simulink model "rfsoc4x2_ospfb_128"  (R2021a)
(part 16 of 339)

      mask prompts: mult_latency "Multiplier Latency"; coeff_width "Coefficient Bit Width In"; coeff_frac_width "Coefficient Fractional Bits"; delay "Data/Sync Delay"; data_width "Data Bit Width In"; bram_latency "BRAM Latency"; use_hdl "Use behavioral HDL for multlipliers"; use_embedded "Use embedded multipliers"
      mask init: same as rfsoc4x2_ospfb_128/pfb_fir_real10/pol1_in1_tap1
  pol1_in1_tap77 : Subsystem  AncestorBlock=casper_library_pfbs/tap_real  mask(pfb_tap_real){mult_latency=2, coeff_width=16, coeff_frac_width=15, delay=16, data_width=16, bram_latency=2, use_hdl=on, use_embedded=off}
      mask prompts: mult_latency "Multiplier Latency"; coeff_width "Coefficient Bit Width In"; coeff_frac_width "Coefficient Fractional Bits"; delay "Data/Sync Delay"; data_width "Data Bit Width In"; bram_latency "BRAM Latency"; use_hdl "Use behavioral HDL for multlipliers"; use_embedded "Use embedded multipliers"
      mask init: same as rfsoc4x2_ospfb_128/pfb_fir_real10/pol1_in1_tap1
  pol1_in1_tap78 : Subsystem  AncestorBlock=casper_library_pfbs/tap_real  mask(pfb_tap_real){mult_latency=2, coeff_width=16, coeff_frac_width=15, delay=16, data_width=16, bram_latency=2, use_hdl=on, use_embedded=off}
      mask prompts: mult_latency "Multiplier Latency"; coeff_width "Coefficient Bit Width In"; coeff_frac_width "Coefficient Fractional Bits"; delay "Data/Sync Delay"; data_width "Data Bit Width In"; bram_latency "BRAM Latency"; use_hdl "Use behavioral HDL for multlipliers"; use_embedded "Use embedded multipliers"
      mask init: same as rfsoc4x2_ospfb_128/pfb_fir_real10/pol1_in1_tap1
  pol1_in1_tap79 : Subsystem  AncestorBlock=casper_library_pfbs/tap_real  mask(pfb_tap_real){mult_latency=2, coeff_width=16, coeff_frac_width=15, delay=16, data_width=16, bram_latency=2, use_hdl=on, use_embedded=off}
      mask prompts: mult_latency "Multiplier Latency"; coeff_width "Coefficient Bit Width In"; coeff_frac_width "Coefficient Fractional Bits"; delay "Data/Sync Delay"; data_width "Data Bit Width In"; bram_latency "BRAM Latency"; use_hdl "Use behavioral HDL for multlipliers"; use_embedded "Use embedded multipliers"
      mask init: same as rfsoc4x2_ospfb_128/pfb_fir_real10/pol1_in1_tap1
  pol1_in1_tap8 : Subsystem  AncestorBlock=casper_library_pfbs/tap_real  mask(pfb_tap_real){mult_latency=2, coeff_width=16, coeff_frac_width=15, delay=16, data_width=16, bram_latency=2, use_hdl=on, use_embedded=off}
      mask prompts: mult_latency "Multiplier Latency"; coeff_width "Coefficient Bit Width In"; coeff_frac_width "Coefficient Fractional Bits"; delay "Data/Sync Delay"; data_width "Data Bit Width In"; bram_latency "BRAM Latency"; use_hdl "Use behavioral HDL for multlipliers"; use_embedded "Use embedded multipliers"
      mask init: same as rfsoc4x2_ospfb_128/pfb_fir_real10/pol1_in1_tap1
  pol1_in1_tap80 : Subsystem  AncestorBlock=casper_library_pfbs/tap_real  mask(pfb_tap_real){mult_latency=2, coeff_width=16, coeff_frac_width=15, delay=16, data_width=16, bram_latency=2, use_hdl=on, use_embedded=off}
      mask prompts: mult_latency "Multiplier Latency"; coeff_width "Coefficient Bit Width In"; coeff_frac_width "Coefficient Fractional Bits"; delay "Data/Sync Delay"; data_width "Data Bit Width In"; bram_latency "BRAM Latency"; use_hdl "Use behavioral HDL for multlipliers"; use_embedded "Use embedded multipliers"
      mask init: same as rfsoc4x2_ospfb_128/pfb_fir_real10/pol1_in1_tap1
  pol1_in1_tap81 : Subsystem  AncestorBlock=casper_library_pfbs/tap_real  mask(pfb_tap_real){mult_latency=2, coeff_width=16, coeff_frac_width=15, delay=16, data_width=16, bram_latency=2, use_hdl=on, use_embedded=off}
      mask prompts: mult_latency "Multiplier Latency"; coeff_width "Coefficient Bit Width In"; coeff_frac_width "Coefficient Fractional Bits"; delay "Data/Sync Delay"; data_width "Data Bit Width In"; bram_latency "BRAM Latency"; use_hdl "Use behavioral HDL for multlipliers"; use_embedded "Use embedded multipliers"
      mask init: same as rfsoc4x2_ospfb_128/pfb_fir_real10/pol1_in1_tap1
  pol1_in1_tap82 : Subsystem  AncestorBlock=casper_library_pfbs/tap_real  mask(pfb_tap_real){mult_latency=2, coeff_width=16, coeff_frac_width=15, delay=16, data_width=16, bram_latency=2, use_hdl=on, use_embedded=off}
      mask prompts: mult_latency "Multiplier Latency"; coeff_width "Coefficient Bit Width In"; coeff_frac_width "Coefficient Fractional Bits"; delay "Data/Sync Delay"; data_width "Data Bit Width In"; bram_latency "BRAM Latency"; use_hdl "Use behavioral HDL for multlipliers"; use_embedded "Use embedded multipliers"
      mask init: same as rfsoc4x2_ospfb_128/pfb_fir_real10/pol1_in1_tap1
  pol1_in1_tap83 : Subsystem  AncestorBlock=casper_library_pfbs/tap_real  mask(pfb_tap_real){mult_latency=2, coeff_width=16, coeff_frac_width=15, delay=16, data_width=16, bram_latency=2, use_hdl=on, use_embedded=off}
      mask prompts: mult_latency "Multiplier Latency"; coeff_width "Coefficient Bit Width In"; coeff_frac_width "Coefficient Fractional Bits"; delay "Data/Sync Delay"; data_width "Data Bit Width In"; bram_latency "BRAM Latency"; use_hdl "Use behavioral HDL for multlipliers"; use_embedded "Use embedded multipliers"
      mask init: same as rfsoc4x2_ospfb_128/pfb_fir_real10/pol1_in1_tap1
  pol1_in1_tap84 : Subsystem  AncestorBlock=casper_library_pfbs/tap_real  mask(pfb_tap_real){mult_latency=2, coeff_width=16, coeff_frac_width=15, delay=16, data_width=16, bram_latency=2, use_hdl=on, use_embedded=off}
      mask prompts: mult_latency "Multiplier Latency"; coeff_width "Coefficient Bit Width In"; coeff_frac_width "Coefficient Fractional Bits"; delay "Data/Sync Delay"; data_width "Data Bit Width In"; bram_latency "BRAM Latency"; use_hdl "Use behavioral HDL for multlipliers"; use_embedded "Use embedded multipliers"
      mask init: same as rfsoc4x2_ospfb_128/pfb_fir_real10/pol1_in1_tap1
  pol1_in1_tap85 : Subsystem  AncestorBlock=casper_library_pfbs/tap_real  mask(pfb_tap_real){mult_latency=2, coeff_width=16, coeff_frac_width=15, delay=16, data_width=16, bram_latency=2, use_hdl=on, use_embedded=off}
      mask prompts: mult_latency "Multiplier Latency"; coeff_width "Coefficient Bit Width In"; coeff_frac_width "Coefficient Fractional Bits"; delay "Data/Sync Delay"; data_width "Data Bit Width In"; bram_latency "BRAM Latency"; use_hdl "Use behavioral HDL for multlipliers"; use_embedded "Use embedded multipliers"
      mask init: same as rfsoc4x2_ospfb_128/pfb_fir_real10/pol1_in1_tap1
  pol1_in1_tap86 : Subsystem  AncestorBlock=casper_library_pfbs/tap_real  mask(pfb_tap_real){mult_latency=2, coeff_width=16, coeff_frac_width=15, delay=16, data_width=16, bram_latency=2, use_hdl=on, use_embedded=off}
      mask prompts: mult_latency "Multiplier Latency"; coeff_width "Coefficient Bit Width In"; coeff_frac_width "Coefficient Fractional Bits"; delay "Data/Sync Delay"; data_width "Data Bit Width In"; bram_latency "BRAM Latency"; use_hdl "Use behavioral HDL for multlipliers"; use_embedded "Use embedded multipliers"
      mask init: same as rfsoc4x2_ospfb_128/pfb_fir_real10/pol1_in1_tap1
  pol1_in1_tap87 : Subsystem  AncestorBlock=casper_library_pfbs/tap_real  mask(pfb_tap_real){mult_latency=2, coeff_width=16, coeff_frac_width=15, delay=16, data_width=16, bram_latency=2, use_hdl=on, use_embedded=off}
      mask prompts: mult_latency "Multiplier Latency"; coeff_width "Coefficient Bit Width In"; coeff_frac_width "Coefficient Fractional Bits"; delay "Data/Sync Delay"; data_width "Data Bit Width In"; bram_latency "BRAM Latency"; use_hdl "Use behavioral HDL for multlipliers"; use_embedded "Use embedded multipliers"
      mask init: same as rfsoc4x2_ospfb_128/pfb_fir_real10/pol1_in1_tap1
  pol1_in1_tap88 : Subsystem  AncestorBlock=casper_library_pfbs/tap_real  mask(pfb_tap_real){mult_latency=2, coeff_width=16, coeff_frac_width=15, delay=16, data_width=16, bram_latency=2, use_hdl=on, use_embedded=off}
      mask prompts: mult_latency "Multiplier Latency"; coeff_width "Coefficient Bit Width In"; coeff_frac_width "Coefficient Fractional Bits"; delay "Data/Sync Delay"; data_width "Data Bit Width In"; bram_latency "BRAM Latency"; use_hdl "Use behavioral HDL for multlipliers"; use_embedded "Use embedded multipliers"
      mask init: same as rfsoc4x2_ospfb_128/pfb_fir_real10/pol1_in1_tap1
  pol1_in1_tap89 : Subsystem  AncestorBlock=casper_library_pfbs/tap_real  mask(pfb_tap_real){mult_latency=2, coeff_width=16, coeff_frac_width=15, delay=16, data_width=16, bram_latency=2, use_hdl=on, use_embedded=off}
      mask prompts: mult_latency "Multiplier Latency"; coeff_width "Coefficient Bit Width In"; coeff_frac_width "Coefficient Fractional Bits"; delay "Data/Sync Delay"; data_width "Data Bit Width In"; bram_latency "BRAM Latency"; use_hdl "Use behavioral HDL for multlipliers"; use_embedded "Use embedded multipliers"
      mask init: same as rfsoc4x2_ospfb_128/pfb_fir_real10/pol1_in1_tap1
  pol1_in1_tap9 : Subsystem  AncestorBlock=casper_library_pfbs/tap_real  mask(pfb_tap_real){mult_latency=2, coeff_width=16, coeff_frac_width=15, delay=16, data_width=16, bram_latency=2, use_hdl=on, use_embedded=off}
      mask prompts: mult_latency "Multiplier Latency"; coeff_width "Coefficient Bit Width In"; coeff_frac_width "Coefficient Fractional Bits"; delay "Data/Sync Delay"; data_width "Data Bit Width In"; bram_latency "BRAM Latency"; use_hdl "Use behavioral HDL for multlipliers"; use_embedded "Use embedded multipliers"
      mask init: same as rfsoc4x2_ospfb_128/pfb_fir_real10/pol1_in1_tap1
  pol1_in1_tap90 : Subsystem  AncestorBlock=casper_library_pfbs/tap_real  mask(pfb_tap_real){mult_latency=2, coeff_width=16, coeff_frac_width=15, delay=16, data_width=16, bram_latency=2, use_hdl=on, use_embedded=off}
      mask prompts: mult_latency "Multiplier Latency"; coeff_width "Coefficient Bit Width In"; coeff_frac_width "Coefficient Fractional Bits"; delay "Data/Sync Delay"; data_width "Data Bit Width In"; bram_latency "BRAM Latency"; use_hdl "Use behavioral HDL for multlipliers"; use_embedded "Use embedded multipliers"
      mask init: same as rfsoc4x2_ospfb_128/pfb_fir_real10/pol1_in1_tap1
  pol1_in1_tap91 : Subsystem  AncestorBlock=casper_library_pfbs/tap_real  mask(pfb_tap_real){mult_latency=2, coeff_width=16, coeff_frac_width=15, delay=16, data_width=16, bram_latency=2, use_hdl=on, use_embedded=off}
      mask prompts: mult_latency "Multiplier Latency"; coeff_width "Coefficient Bit Width In"; coeff_frac_width "Coefficient Fractional Bits"; delay "Data/Sync Delay"; data_width "Data Bit Width In"; bram_latency "BRAM Latency"; use_hdl "Use behavioral HDL for multlipliers"; use_embedded "Use embedded multipliers"
      mask init: same as rfsoc4x2_ospfb_128/pfb_fir_real10/pol1_in1_tap1
  pol1_in1_tap92 : Subsystem  AncestorBlock=casper_library_pfbs/tap_real  mask(pfb_tap_real){mult_latency=2, coeff_width=16, coeff_frac_width=15, delay=16, data_width=16, bram_latency=2, use_hdl=on, use_embedded=off}
      mask prompts: mult_latency "Multiplier Latency"; coeff_width "Coefficient Bit Width In"; coeff_frac_width "Coefficient Fractional Bits"; delay "Data/Sync Delay"; data_width "Data Bit Width In"; bram_latency "BRAM Latency"; use_hdl "Use behavioral HDL for multlipliers"; use_embedded "Use embedded multipliers"
      mask init: same as rfsoc4x2_ospfb_128/pfb_fir_real10/pol1_in1_tap1
  pol1_in1_tap93 : Subsystem  AncestorBlock=casper_library_pfbs/tap_real  mask(pfb_tap_real){mult_latency=2, coeff_width=16, coeff_frac_width=15, delay=16, data_width=16, bram_latency=2, use_hdl=on, use_embedded=off}
      mask prompts: mult_latency "Multiplier Latency"; coeff_width "Coefficient Bit Width In"; coeff_frac_width "Coefficient Fractional Bits"; delay "Data/Sync Delay"; data_width "Data Bit Width In"; bram_latency "BRAM Latency"; use_hdl "Use behavioral HDL for multlipliers"; use_embedded "Use embedded multipliers"
      mask init: same as rfsoc4x2_ospfb_128/pfb_fir_real10/pol1_in1_tap1
  pol1_in1_tap94 : Subsystem  AncestorBlock=casper_library_pfbs/tap_real  mask(pfb_tap_real){mult_latency=2, coeff_width=16, coeff_frac_width=15, delay=16, data_width=16, bram_latency=2, use_hdl=on, use_embedded=off}
      mask prompts: mult_latency "Multiplier Latency"; coeff_width "Coefficient Bit Width In"; coeff_frac_width "Coefficient Fractional Bits"; delay "Data/Sync Delay"; data_width "Data Bit Width In"; bram_latency "BRAM Latency"; use_hdl "Use behavioral HDL for multlipliers"; use_embedded "Use embedded multipliers"
      mask init: same as rfsoc4x2_ospfb_128/pfb_fir_real10/pol1_in1_tap1
  pol1_in1_tap95 : Subsystem  AncestorBlock=casper_library_pfbs/tap_real  mask(pfb_tap_real){mult_latency=2, coeff_width=16, coeff_frac_width=15, delay=16, data_width=16, bram_latency=2, use_hdl=on, use_embedded=off}
      mask prompts: mult_latency "Multiplier Latency"; coeff_width "Coefficient Bit Width In"; coeff_frac_width "Coefficient Fractional Bits"; delay "Data/Sync Delay"; data_width "Data Bit Width In"; bram_latency "BRAM Latency"; use_hdl "Use behavioral HDL for multlipliers"; use_embedded "Use embedded multipliers"
      mask init: same as rfsoc4x2_ospfb_128/pfb_fir_real10/pol1_in1_tap1
  pol1_in1_tap96 : Subsystem  AncestorBlock=casper_library_pfbs/tap_real  mask(pfb_tap_real){mult_latency=2, coeff_width=16, coeff_frac_width=15, delay=16, data_width=16, bram_latency=2, use_hdl=on, use_embedded=off}
      mask prompts: mult_latency "Multiplier Latency"; coeff_width "Coefficient Bit Width In"; coeff_frac_width "Coefficient Fractional Bits"; delay "Data/Sync Delay"; data_width "Data Bit Width In"; bram_latency "BRAM Latency"; use_hdl "Use behavioral HDL for multlipliers"; use_embedded "Use embedded multipliers"
      mask init: same as rfsoc4x2_ospfb_128/pfb_fir_real10/pol1_in1_tap1
  pol1_in2_coeffs : Subsystem  AncestorBlock=casper_library_pfbs/pfb_coeff_gen  mask(pfb_coeff_gen){PFBSize=8, CoeffBitWidth=16, TotalTaps=8, CoeffDistMem=off, WindowType=hamming, bram_latency=2, n_inputs=4, nput=1, fwidth=1.245000000000000106581410364015, debug_mode=off, fan_latency=1}
      mask prompts: PFBSize "Size of PFB: (2^? pnts)"; CoeffBitWidth "Bitwidth of Coefficients:"; TotalTaps "Total Number of Taps:"; CoeffDistMem "Implement Coeff Gen in Distributed Memory"; WindowType "Windowing Function:"; bram_latency "BRAM Latency"; n_inputs "Number of Simultaneous Inputs: (2^?)"; nput "This is input number:"; fwidth "Bin Width (normal=1)"; debug_mode "Debug mode - coeffs are a [1:pfb_size*taps] ramp."; fan_latency "Fanout latency"
      mask init: same as rfsoc4x2_ospfb_128/pfb_fir_real10/pol1_in10_coeffs
      settings: AttributesFormatString=|
      | PFBSize=8, n_inputs=4,
      | taps=8, input=1
  pol1_in3_coeffs : Subsystem  AncestorBlock=casper_library_pfbs/pfb_coeff_gen  mask(pfb_coeff_gen){PFBSize=8, CoeffBitWidth=16, TotalTaps=8, CoeffDistMem=off, WindowType=hamming, bram_latency=2, n_inputs=4, nput=2, fwidth=1.245000000000000106581410364015, debug_mode=off, fan_latency=1}
      mask prompts: PFBSize "Size of PFB: (2^? pnts)"; CoeffBitWidth "Bitwidth of Coefficients:"; TotalTaps "Total Number of Taps:"; CoeffDistMem "Implement Coeff Gen in Distributed Memory"; WindowType "Windowing Function:"; bram_latency "BRAM Latency"; n_inputs "Number of Simultaneous Inputs: (2^?)"; nput "This is input number:"; fwidth "Bin Width (normal=1)"; debug_mode "Debug mode - coeffs are a [1:pfb_size*taps] ramp."; fan_latency "Fanout latency"
      mask init: same as rfsoc4x2_ospfb_128/pfb_fir_real10/pol1_in10_coeffs
      settings: AttributesFormatString=|
      | PFBSize=8, n_inputs=4,
      | taps=8, input=2
  pol1_in4_coeffs : Subsystem  AncestorBlock=casper_library_pfbs/pfb_coeff_gen  mask(pfb_coeff_gen){PFBSize=8, CoeffBitWidth=16, TotalTaps=8, CoeffDistMem=off, WindowType=hamming, bram_latency=2, n_inputs=4, nput=3, fwidth=1.245000000000000106581410364015, debug_mode=off, fan_latency=1}
      mask prompts: PFBSize "Size of PFB: (2^? pnts)"; CoeffBitWidth "Bitwidth of Coefficients:"; TotalTaps "Total Number of Taps:"; CoeffDistMem "Implement Coeff Gen in Distributed Memory"; WindowType "Windowing Function:"; bram_latency "BRAM Latency"; n_inputs "Number of Simultaneous Inputs: (2^?)"; nput "This is input number:"; fwidth "Bin Width (normal=1)"; debug_mode "Debug mode - coeffs are a [1:pfb_size*taps] ramp."; fan_latency "Fanout latency"
      mask init: same as rfsoc4x2_ospfb_128/pfb_fir_real10/pol1_in10_coeffs
      settings: AttributesFormatString=|
      | PFBSize=8, n_inputs=4,
      | taps=8, input=3
  pol1_in5_coeffs : Subsystem  AncestorBlock=casper_library_pfbs/pfb_coeff_gen  mask(pfb_coeff_gen){PFBSize=8, CoeffBitWidth=16, TotalTaps=8, CoeffDistMem=off, WindowType=hamming, bram_latency=2, n_inputs=4, nput=4, fwidth=1.245000000000000106581410364015, debug_mode=off, fan_latency=1}
      mask prompts: PFBSize "Size of PFB: (2^? pnts)"; CoeffBitWidth "Bitwidth of Coefficients:"; TotalTaps "Total Number of Taps:"; CoeffDistMem "Implement Coeff Gen in Distributed Memory"; WindowType "Windowing Function:"; bram_latency "BRAM Latency"; n_inputs "Number of Simultaneous Inputs: (2^?)"; nput "This is input number:"; fwidth "Bin Width (normal=1)"; debug_mode "Debug mode - coeffs are a [1:pfb_size*taps] ramp."; fan_latency "Fanout latency"
      mask init: same as rfsoc4x2_ospfb_128/pfb_fir_real10/pol1_in10_coeffs
      settings: AttributesFormatString=|
      | PFBSize=8, n_inputs=4,
      | taps=8, input=4
  pol1_in6_coeffs : Subsystem  AncestorBlock=casper_library_pfbs/pfb_coeff_gen  mask(pfb_coeff_gen){PFBSize=8, CoeffBitWidth=16, TotalTaps=8, CoeffDistMem=off, WindowType=hamming, bram_latency=2, n_inputs=4, nput=5, fwidth=1.245000000000000106581410364015, debug_mode=off, fan_latency=1}
      mask prompts: PFBSize "Size of PFB: (2^? pnts)"; CoeffBitWidth "Bitwidth of Coefficients:"; TotalTaps "Total Number of Taps:"; CoeffDistMem "Implement Coeff Gen in Distributed Memory"; WindowType "Windowing Function:"; bram_latency "BRAM Latency"; n_inputs "Number of Simultaneous Inputs: (2^?)"; nput "This is input number:"; fwidth "Bin Width (normal=1)"; debug_mode "Debug mode - coeffs are a [1:pfb_size*taps] ramp."; fan_latency "Fanout latency"
      mask init: same as rfsoc4x2_ospfb_128/pfb_fir_real10/pol1_in10_coeffs
      settings: AttributesFormatString=|
      | PFBSize=8, n_inputs=4,
      | taps=8, input=5
  pol1_in7_coeffs : Subsystem  AncestorBlock=casper_library_pfbs/pfb_coeff_gen  mask(pfb_coeff_gen){PFBSize=8, CoeffBitWidth=16, TotalTaps=8, CoeffDistMem=off, WindowType=hamming, bram_latency=2, n_inputs=4, nput=6, fwidth=1.245000000000000106581410364015, debug_mode=off, fan_latency=1}
      mask prompts: PFBSize "Size of PFB: (2^? pnts)"; CoeffBitWidth "Bitwidth of Coefficients:"; TotalTaps "Total Number of Taps:"; CoeffDistMem "Implement Coeff Gen in Distributed Memory"; WindowType "Windowing Function:"; bram_latency "BRAM Latency"; n_inputs "Number of Simultaneous Inputs: (2^?)"; nput "This is input number:"; fwidth "Bin Width (normal=1)"; debug_mode "Debug mode - coeffs are a [1:pfb_size*taps] ramp."; fan_latency "Fanout latency"
      mask init: same as rfsoc4x2_ospfb_128/pfb_fir_real10/pol1_in10_coeffs
      settings: AttributesFormatString=|
      | PFBSize=8, n_inputs=4,
      | taps=8, input=6
  pol1_in8_coeffs : Subsystem  AncestorBlock=casper_library_pfbs/pfb_coeff_gen  mask(pfb_coeff_gen){PFBSize=8, CoeffBitWidth=16, TotalTaps=8, CoeffDistMem=off, WindowType=hamming, bram_latency=2, n_inputs=4, nput=7, fwidth=1.245000000000000106581410364015, debug_mode=off, fan_latency=1}
      mask prompts: PFBSize "Size of PFB: (2^? pnts)"; CoeffBitWidth "Bitwidth of Coefficients:"; TotalTaps "Total Number of Taps:"; CoeffDistMem "Implement Coeff Gen in Distributed Memory"; WindowType "Windowing Function:"; bram_latency "BRAM Latency"; n_inputs "Number of Simultaneous Inputs: (2^?)"; nput "This is input number:"; fwidth "Bin Width (normal=1)"; debug_mode "Debug mode - coeffs are a [1:pfb_size*taps] ramp."; fan_latency "Fanout latency"
      mask init: same as rfsoc4x2_ospfb_128/pfb_fir_real10/pol1_in10_coeffs
      settings: AttributesFormatString=|
      | PFBSize=8, n_inputs=4,
      | taps=8, input=7
  pol1_in9_coeffs : Subsystem  AncestorBlock=casper_library_pfbs/pfb_coeff_gen  mask(pfb_coeff_gen){PFBSize=8, CoeffBitWidth=16, TotalTaps=8, CoeffDistMem=off, WindowType=hamming, bram_latency=2, n_inputs=4, nput=8, fwidth=1.245000000000000106581410364015, debug_mode=off, fan_latency=1}
      mask prompts: PFBSize "Size of PFB: (2^? pnts)"; CoeffBitWidth "Bitwidth of Coefficients:"; TotalTaps "Total Number of Taps:"; CoeffDistMem "Implement Coeff Gen in Distributed Memory"; WindowType "Windowing Function:"; bram_latency "BRAM Latency"; n_inputs "Number of Simultaneous Inputs: (2^?)"; nput "This is input number:"; fwidth "Bin Width (normal=1)"; debug_mode "Debug mode - coeffs are a [1:pfb_size*taps] ramp."; fan_latency "Fanout latency"
      mask init: same as rfsoc4x2_ospfb_128/pfb_fir_real10/pol1_in10_coeffs
      settings: AttributesFormatString=|
      | PFBSize=8, n_inputs=4,
      | taps=8, input=8
  scale_1_{1..16} (16 alike) : xbsIndex_r4/Scale  scale_factor=-1  dbl_ovrd=off  block_type=scale
  scope{85..86,88..90} (5 alike) : Scope
  sync_out : Outport  VectorParamsAs1DForOutWhenUnconnected=off
  pol1_out1 : Outport  Port=2  VectorParamsAs1DForOutWhenUnconnected=off
  pol1_out2 : Outport  Port=3  VectorParamsAs1DForOutWhenUnconnected=off
  pol1_out3 : Outport  Port=4
  pol1_out4 : Outport  Port=5
  pol1_out5 : Outport  Port=6
  pol1_out6 : Outport  Port=7
  pol1_out7 : Outport  Port=8
  pol1_out8 : Outport  Port=9
  pol1_out9 : Outport  Port=10
  pol1_out10 : Outport  Port=11
  pol1_out11 : Outport  Port=12
  pol1_out12 : Outport  Port=13
  pol1_out13 : Outport  Port=14
  pol1_out14 : Outport  Port=15
  pol1_out15 : Outport  Port=16
  pol1_out16 : Outport  Port=17
  wires:
  pol1_in1_last_tap/1(tap_out) -> adder_1_1/9(din8)
  delay25/1 -> adder_1_1/1(sync)
  pol1_in1_last_tap/2(sync_out) -> delay25/1
  delay24/1 -> adder_1_1/2(din1)
  delay23/1 -> adder_1_1/3(din2)
  delay22/1 -> adder_1_1/4(din3)
  delay21/1 -> adder_1_1/5(din4)
  delay20/1 -> adder_1_1/6(din5)
  delay19/1 -> adder_1_1/7(din6)
  delay18/1 -> adder_1_1/8(din7)
  pol1_in1_tap3/1(dout) -> pol1_in1_tap4/1(din)
  pol1_in1_tap6/6(pot_en_out) -> pol1_in1_tap7/5(pot_en_in)
  pol1_in1_tap6/5(add_out) -> pol1_in1_tap7/4(addr_in)
  pol1_in1_tap5/6(pot_en_out) -> pol1_in1_tap6/5(pot_en_in)
  pol1_in1_tap5/5(add_out) -> pol1_in1_tap6/4(addr_in)
  pol1_in1_tap4/6(pot_en_out) -> pol1_in1_tap5/5(pot_en_in)
  pol1_in1_tap4/5(add_out) -> pol1_in1_tap5/4(addr_in)
  pol1_in1_tap3/6(pot_en_out) -> pol1_in1_tap4/5(pot_en_in)
  pol1_in1_tap3/5(add_out) -> pol1_in1_tap4/4(addr_in)
  pol1_in1_tap2/6(pot_en_out) -> pol1_in1_tap3/5(pot_en_in)
  pol1_in1_tap2/5(add_out) -> pol1_in1_tap3/4(addr_in)
  pol1_in1_first_tap/6(pot_en_out) -> pol1_in1_tap2/5(pot_en_in)
  pol1_in1_first_tap/5(add_out) -> pol1_in1_tap2/4(addr_in)
  [tap_write_en] -> pol1_in1_first_tap/5(pot_en_in)
  [addr] -> pol1_in1_first_tap/4(addr_in)
  Inverter/1 -> [tap_write_en], Gateway Out255/1
  sync/1 -> pol1_in16_coeffs/2(sync), pol1_in15_coeffs/2(sync), pol1_in14_coeffs/2(sync), pol1_in13_coeffs/2(sync), pol1_in12_coeffs/2(sync), pol1_in11_coeffs/2(sync), pol1_in10_coeffs/2(sync), pol1_in9_coeffs/2(sync), pol1_in8_coeffs/2(sync), pol1_in7_coeffs/2(sync), pol1_in6_coeffs/2(sync), pol1_in5_coeffs/2(sync), pol1_in4_coeffs/2(sync), pol1_in3_coeffs/2(sync), pol1_in2_coeffs/2(sync), pol1_in1_coeffs/2(sync), delay2/1
  AddSub12/1 -> Mux3/3
  Mux3/1 -> [addr], Gateway Out251/1
  edge_detect8/1(out) -> Logical11/2
  Delay27/1 -> Logical11/1
  Counter36/1 -> AddSub11/2, Gateway Out253/1
  Constant61/1 -> Relational11/2
  Constant63/1 -> Relational12/2
  Slice20/1 -> edge_detect8/1(in)
  AddSub11/1 -> AddSub12/1, Mux3/2, Relational11/1, Gateway Out250/1
  Constant62/1 -> AddSub12/2
  Counter38/1 -> Slice20/1, Delay26/1
  Relational11/1 -> Mux3/1
  delay2/1 -> Counter36/1, Counter38/1
  Relational12/1 -> Inverter/1
  Delay26/1 -> Relational12/1, AddSub11/1, Gateway Out252/1
  Logical11/1 -> Counter36/2
  Gateway Out251/1 -> scope86/1
  Gateway Out255/1 -> scope90/1
  Gateway Out250/1 -> scope89/1
  en_ctrl/1 -> Delay27/1
  Gateway Out253/1 -> scope85/1
  Gateway Out252/1 -> scope88/1
  pol1_in1_tap7/4(taps_out) -> delay18/1
  pol1_in1_tap7/3(coeff_out) -> pol1_in1_last_tap/3(coeff)
  pol1_in1_tap7/2(sync_out) -> pol1_in1_last_tap/2(sync)
  pol1_in1_tap7/1(dout) -> pol1_in1_last_tap/1(din)
  pol1_in1_tap6/4(taps_out) -> delay19/1
  pol1_in1_tap6/3(coeff_out) -> pol1_in1_tap7/3(coeff)
  pol1_in1_tap6/2(sync_out) -> pol1_in1_tap7/2(sync)
  pol1_in1_tap6/1(dout) -> pol1_in1_tap7/1(din)
  pol1_in1_tap5/4(taps_out) -> delay20/1
  pol1_in1_tap5/3(coeff_out) -> pol1_in1_tap6/3(coeff)
  pol1_in1_tap5/2(sync_out) -> pol1_in1_tap6/2(sync)
  pol1_in1_tap5/1(dout) -> pol1_in1_tap6/1(din)
  pol1_in1_tap4/4(taps_out) -> delay21/1
  pol1_in1_tap4/3(coeff_out) -> pol1_in1_tap5/3(coeff)
  pol1_in1_tap4/2(sync_out) -> pol1_in1_tap5/2(sync)
  pol1_in1_tap4/1(dout) -> pol1_in1_tap5/1(din)
  pol1_in1_tap3/4(taps_out) -> delay22/1
  pol1_in1_tap3/3(coeff_out) -> pol1_in1_tap4/3(coeff)
  pol1_in1_tap3/2(sync_out) -> pol1_in1_tap4/2(sync)
  pol1_in1_tap2/4(taps_out) -> delay23/1
  pol1_in1_tap2/3(coeff_out) -> pol1_in1_tap3/3(coeff)
  pol1_in1_tap2/2(sync_out) -> pol1_in1_tap3/2(sync)
  pol1_in1_tap2/1(dout) -> pol1_in1_tap3/1(din)
  pol1_in1_first_tap/4(taps_out) -> delay24/1
  pol1_in1_first_tap/3(coeff_out) -> pol1_in1_tap2/3(coeff)
  pol1_in1_first_tap/2(sync_out) -> pol1_in1_tap2/2(sync)
  pol1_in1_first_tap/1(dout) -> pol1_in1_tap2/1(din)
  convert_1_16/1 -> pol1_out16/1
  scale_1_16/1 -> convert_1_16/1
  adder_1_16/2(dout) -> scale_1_16/1
  convert_1_15/1 -> pol1_out15/1
  scale_1_15/1 -> convert_1_15/1
  adder_1_15/2(dout) -> scale_1_15/1
  convert_1_14/1 -> pol1_out14/1
  scale_1_14/1 -> convert_1_14/1
  adder_1_14/2(dout) -> scale_1_14/1
  convert_1_13/1 -> pol1_out13/1
  scale_1_13/1 -> convert_1_13/1
  adder_1_13/2(dout) -> scale_1_13/1
  convert_1_12/1 -> pol1_out12/1
  scale_1_12/1 -> convert_1_12/1
  adder_1_12/2(dout) -> scale_1_12/1
  convert_1_11/1 -> pol1_out11/1
  scale_1_11/1 -> convert_1_11/1
  adder_1_11/2(dout) -> scale_1_11/1
  convert_1_10/1 -> pol1_out10/1
  scale_1_10/1 -> convert_1_10/1
  adder_1_10/2(dout) -> scale_1_10/1
  convert_1_9/1 -> pol1_out9/1
  scale_1_9/1 -> convert_1_9/1
  adder_1_9/2(dout) -> scale_1_9/1
  convert_1_8/1 -> pol1_out8/1
  scale_1_8/1 -> convert_1_8/1
  adder_1_8/2(dout) -> scale_1_8/1
  convert_1_7/1 -> pol1_out7/1
  scale_1_7/1 -> convert_1_7/1
  adder_1_7/2(dout) -> scale_1_7/1
  convert_1_6/1 -> pol1_out6/1
  scale_1_6/1 -> convert_1_6/1
  adder_1_6/2(dout) -> scale_1_6/1
  convert_1_5/1 -> pol1_out5/1
  scale_1_5/1 -> convert_1_5/1
  adder_1_5/2(dout) -> scale_1_5/1
  convert_1_4/1 -> pol1_out4/1
  scale_1_4/1 -> convert_1_4/1
  adder_1_4/2(dout) -> scale_1_4/1
  convert_1_3/1 -> pol1_out3/1
  scale_1_3/1 -> convert_1_3/1
  adder_1_3/2(dout) -> scale_1_3/1
  convert_1_2/1 -> pol1_out2/1
  scale_1_2/1 -> convert_1_2/1
  adder_1_2/2(dout) -> scale_1_2/1
  convert_1_1/1 -> pol1_out1/1
  scale_1_1/1 -> convert_1_1/1
  adder_1_1/2(dout) -> scale_1_1/1
  delay1/1 -> sync_out/1
  adder_1_1/1(sync_out) -> delay1/1
  pol1_in16/1 -> pol1_in16_coeffs/1(din)
  pol1_in15/1 -> pol1_in15_coeffs/1(din)
  pol1_in14/1 -> pol1_in14_coeffs/1(din)
  pol1_in13/1 -> pol1_in13_coeffs/1(din)
  pol1_in12/1 -> pol1_in12_coeffs/1(din)
  pol1_in11/1 -> pol1_in11_coeffs/1(din)
  pol1_in10/1 -> pol1_in10_coeffs/1(din)
  pol1_in9/1 -> pol1_in9_coeffs/1(din)
  pol1_in8/1 -> pol1_in8_coeffs/1(din)
  pol1_in7/1 -> pol1_in7_coeffs/1(din)
  pol1_in6/1 -> pol1_in6_coeffs/1(din)
  pol1_in5/1 -> pol1_in5_coeffs/1(din)
  pol1_in4/1 -> pol1_in4_coeffs/1(din)
  pol1_in3/1 -> pol1_in3_coeffs/1(din)
  pol1_in2/1 -> pol1_in2_coeffs/1(din)
  pol1_in1_coeffs/3(coeff) -> pol1_in1_first_tap/3(coeffs)
  pol1_in1_coeffs/1(dout) -> pol1_in1_first_tap/1(din)
  pol1_in1/1 -> pol1_in1_coeffs/1(din)
  pol1_in1_coeffs/2(sync_out) -> pol1_in1_first_tap/2(sync)
  pol1_in1_first_tap1/1(dout) -> pol1_in1_tap1/1(din)
  pol1_in1_first_tap1/2(sync_out) -> pol1_in1_tap1/2(sync)
  pol1_in1_first_tap1/3(coeff_out) -> pol1_in1_tap1/3(coeff)
  pol1_in1_first_tap1/4(taps_out) -> delay9/1
  pol1_in1_tap1/1(dout) -> pol1_in1_tap8/1(din)
  pol1_in1_tap1/2(sync_out) -> pol1_in1_tap8/2(sync)
  pol1_in1_tap1/3(coeff_out) -> pol1_in1_tap8/3(coeff)
  pol1_in1_tap1/4(taps_out) -> delay8/1
  pol1_in1_tap8/2(sync_out) -> pol1_in1_tap9/2(sync)
  pol1_in1_tap8/3(coeff_out) -> pol1_in1_tap9/3(coeff)
  pol1_in1_tap8/4(taps_out) -> delay7/1
  pol1_in1_tap9/1(dout) -> pol1_in1_tap10/1(din)
  pol1_in1_tap9/2(sync_out) -> pol1_in1_tap10/2(sync)
  pol1_in1_tap9/3(coeff_out) -> pol1_in1_tap10/3(coeff)
  pol1_in1_tap9/4(taps_out) -> delay6/1
  pol1_in1_tap10/1(dout) -> pol1_in1_tap11/1(din)
  pol1_in1_tap10/2(sync_out) -> pol1_in1_tap11/2(sync)
  pol1_in1_tap10/3(coeff_out) -> pol1_in1_tap11/3(coeff)
  pol1_in1_tap10/4(taps_out) -> delay5/1
  pol1_in1_tap11/1(dout) -> pol1_in1_tap12/1(din)
  pol1_in1_tap11/2(sync_out) -> pol1_in1_tap12/2(sync)
  pol1_in1_tap11/3(coeff_out) -> pol1_in1_tap12/3(coeff)
  pol1_in1_tap11/4(taps_out) -> delay4/1
  pol1_in1_tap12/1(dout) -> pol1_in1_last_tap1/1(din)
  pol1_in1_tap12/2(sync_out) -> pol1_in1_last_tap1/2(sync)
  pol1_in1_tap12/3(coeff_out) -> pol1_in1_last_tap1/3(coeff)
  pol1_in1_tap12/4(taps_out) -> delay3/1
  pol1_in1_first_tap1/5(add_out) -> pol1_in1_tap1/4(addr_in)
  pol1_in1_first_tap1/6(pot_en_out) -> pol1_in1_tap1/5(pot_en_in)
  pol1_in1_tap1/5(add_out) -> pol1_in1_tap8/4(addr_in)
  pol1_in1_tap1/6(pot_en_out) -> pol1_in1_tap8/5(pot_en_in)
  pol1_in1_tap8/5(add_out) -> pol1_in1_tap9/4(addr_in)
  pol1_in1_tap8/6(pot_en_out) -> pol1_in1_tap9/5(pot_en_in)
  pol1_in1_tap9/5(add_out) -> pol1_in1_tap10/4(addr_in)
  pol1_in1_tap9/6(pot_en_out) -> pol1_in1_tap10/5(pot_en_in)
  pol1_in1_tap10/5(add_out) -> pol1_in1_tap11/4(addr_in)
  pol1_in1_tap10/6(pot_en_out) -> pol1_in1_tap11/5(pot_en_in)
  pol1_in1_tap11/5(add_out) -> pol1_in1_tap12/4(addr_in)
  pol1_in1_tap11/6(pot_en_out) -> pol1_in1_tap12/5(pot_en_in)
  pol1_in1_tap8/1(dout) -> pol1_in1_tap9/1(din)
  delay3/1 -> adder_1_2/8(din7)
  delay4/1 -> adder_1_2/7(din6)
  delay5/1 -> adder_1_2/6(din5)
  delay6/1 -> adder_1_2/5(din4)
  delay7/1 -> adder_1_2/4(din3)
  delay8/1 -> adder_1_2/3(din2)
  delay9/1 -> adder_1_2/2(din1)
  pol1_in1_last_tap1/2(sync_out) -> delay10/1
  delay10/1 -> adder_1_2/1(sync)
  pol1_in1_last_tap1/1(tap_out) -> adder_1_2/9(din8)
  pol1_in2_coeffs/1(dout) -> pol1_in1_first_tap1/1(din)
  pol1_in2_coeffs/3(coeff) -> pol1_in1_first_tap1/3(coeffs)
  [addr] -> pol1_in1_first_tap1/4(addr_in)
  [tap_write_en] -> pol1_in1_first_tap1/5(pot_en_in)
  pol1_in1_tap15/3(coeff_out) -> pol1_in1_tap16/3(coeff)
  pol1_in1_tap17/5(add_out) -> pol1_in1_tap18/4(addr_in)
  pol1_in1_first_tap2/6(pot_en_out) -> pol1_in1_tap13/5(pot_en_in)
  pol1_in1_tap16/3(coeff_out) -> pol1_in1_last_tap2/3(coeff)
  pol1_in1_tap14/4(taps_out) -> delay14/1
  pol1_in1_tap15/2(sync_out) -> pol1_in1_tap16/2(sync)
  [tap_write_en] -> pol1_in1_first_tap2/5(pot_en_in)
  pol1_in1_tap18/1(dout) -> pol1_in1_tap14/1(din)
  pol1_in1_tap18/5(add_out) -> pol1_in1_tap14/4(addr_in)
  pol1_in1_tap13/6(pot_en_out) -> pol1_in1_tap17/5(pot_en_in)
  pol1_in1_tap14/5(add_out) -> pol1_in1_tap15/4(addr_in)
  pol1_in1_last_tap2/1(tap_out) -> adder_1_3/9(din8)
  pol1_in1_first_tap2/4(taps_out) -> delay26/1
  pol1_in1_tap17/1(dout) -> pol1_in1_tap18/1(din)
  pol1_in1_tap14/2(sync_out) -> pol1_in1_tap15/2(sync)
  pol1_in3_coeffs/3(coeff) -> pol1_in1_first_tap2/3(coeffs)
  pol1_in1_tap16/1(dout) -> pol1_in1_last_tap2/1(din)
  [addr] -> pol1_in1_first_tap2/4(addr_in)
  pol1_in1_tap15/1(dout) -> pol1_in1_tap16/1(din)
  pol1_in1_tap17/3(coeff_out) -> pol1_in1_tap18/3(coeff)
  pol1_in1_tap13/3(coeff_out) -> pol1_in1_tap17/3(coeff)
  pol1_in1_tap13/1(dout) -> pol1_in1_tap17/1(din)
  delay16/1 -> adder_1_3/4(din3)
  pol1_in1_tap18/3(coeff_out) -> pol1_in1_tap14/3(coeff)
  pol1_in1_tap13/5(add_out) -> pol1_in1_tap17/4(addr_in)
  pol1_in1_tap14/1(dout) -> pol1_in1_tap15/1(din)
  pol1_in1_tap14/6(pot_en_out) -> pol1_in1_tap15/5(pot_en_in)
  pol1_in1_tap17/2(sync_out) -> pol1_in1_tap18/2(sync)
  pol1_in1_tap13/2(sync_out) -> pol1_in1_tap17/2(sync)
  pol1_in1_first_tap2/3(coeff_out) -> pol1_in1_tap13/3(coeff)
  pol1_in1_last_tap2/2(sync_out) -> delay11/1
  pol1_in1_tap17/4(taps_out) -> delay16/1
  pol1_in1_tap13/4(taps_out) -> delay17/1
  pol1_in1_tap16/4(taps_out) -> delay12/1
  pol1_in1_tap15/6(pot_en_out) -> pol1_in1_tap16/5(pot_en_in)
  delay12/1 -> adder_1_3/8(din7)
  pol1_in1_first_tap2/5(add_out) -> pol1_in1_tap13/4(addr_in)
  pol1_in1_tap18/2(sync_out) -> pol1_in1_tap14/2(sync)
  delay11/1 -> adder_1_3/1(sync)
  pol1_in1_tap14/3(coeff_out) -> pol1_in1_tap15/3(coeff)
  pol1_in1_first_tap2/1(dout) -> pol1_in1_tap13/1(din)
  pol1_in1_tap18/4(taps_out) -> delay15/1
  delay26/1 -> adder_1_3/2(din1)
  pol1_in1_tap15/5(add_out) -> pol1_in1_tap16/4(addr_in)
  delay13/1 -> adder_1_3/7(din6)
  delay14/1 -> adder_1_3/6(din5)
  pol1_in1_tap16/2(sync_out) -> pol1_in1_last_tap2/2(sync)
  pol1_in1_tap18/6(pot_en_out) -> pol1_in1_tap14/5(pot_en_in)
  pol1_in1_tap17/6(pot_en_out) -> pol1_in1_tap18/5(pot_en_in)
  pol1_in1_first_tap2/2(sync_out) -> pol1_in1_tap13/2(sync)
  pol1_in1_tap15/4(taps_out) -> delay13/1
  delay15/1 -> adder_1_3/5(din4)
  delay17/1 -> adder_1_3/3(din2)
  pol1_in3_coeffs/1(dout) -> pol1_in1_first_tap2/1(din)
  pol1_in1_tap21/3(coeff_out) -> pol1_in1_tap22/3(coeff)
  pol1_in1_tap23/5(add_out) -> pol1_in1_tap24/4(addr_in)
  pol1_in1_first_tap3/6(pot_en_out) -> pol1_in1_tap19/5(pot_en_in)
  pol1_in1_tap22/3(coeff_out) -> pol1_in1_last_tap3/3(coeff)
  pol1_in1_tap20/4(taps_out) -> delay30/1
  pol1_in1_tap21/2(sync_out) -> pol1_in1_tap22/2(sync)
  [tap_write_en] -> pol1_in1_first_tap3/5(pot_en_in)
  pol1_in1_tap24/1(dout) -> pol1_in1_tap20/1(din)
  pol1_in1_tap24/5(add_out) -> pol1_in1_tap20/4(addr_in)
  pol1_in1_tap19/6(pot_en_out) -> pol1_in1_tap23/5(pot_en_in)
  pol1_in1_tap20/5(add_out) -> pol1_in1_tap21/4(addr_in)
  pol1_in1_last_tap3/1(tap_out) -> adder_1_4/9(din8)
  pol1_in1_first_tap3/4(taps_out) -> delay34/1
  pol1_in1_tap23/1(dout) -> pol1_in1_tap24/1(din)
  pol1_in1_tap20/2(sync_out) -> pol1_in1_tap21/2(sync)
  pol1_in4_coeffs/3(coeff) -> pol1_in1_first_tap3/3(coeffs)
  pol1_in1_tap22/1(dout) -> pol1_in1_last_tap3/1(din)
  [addr] -> pol1_in1_first_tap3/4(addr_in)
  pol1_in1_tap21/1(dout) -> pol1_in1_tap22/1(din)
  pol1_in1_tap23/3(coeff_out) -> pol1_in1_tap24/3(coeff)
  pol1_in1_tap19/3(coeff_out) -> pol1_in1_tap23/3(coeff)
  pol1_in1_tap19/1(dout) -> pol1_in1_tap23/1(din)
  delay32/1 -> adder_1_4/4(din3)
  pol1_in1_tap24/3(coeff_out) -> pol1_in1_tap20/3(coeff)
  pol1_in1_tap19/5(add_out) -> pol1_in1_tap23/4(addr_in)
  pol1_in1_tap20/1(dout) -> pol1_in1_tap21/1(din)
  pol1_in1_tap20/6(pot_en_out) -> pol1_in1_tap21/5(pot_en_in)
  pol1_in1_tap23/2(sync_out) -> pol1_in1_tap24/2(sync)
  pol1_in1_tap19/2(sync_out) -> pol1_in1_tap23/2(sync)
  pol1_in1_first_tap3/3(coeff_out) -> pol1_in1_tap19/3(coeff)
  pol1_in1_last_tap3/2(sync_out) -> delay27/1
  pol1_in1_tap23/4(taps_out) -> delay32/1
  pol1_in1_tap19/4(taps_out) -> delay33/1
  pol1_in1_tap22/4(taps_out) -> delay28/1
  pol1_in1_tap21/6(pot_en_out) -> pol1_in1_tap22/5(pot_en_in)
  delay28/1 -> adder_1_4/8(din7)
  pol1_in1_first_tap3/5(add_out) -> pol1_in1_tap19/4(addr_in)
  pol1_in1_tap24/2(sync_out) -> pol1_in1_tap20/2(sync)
  delay27/1 -> adder_1_4/1(sync)
  pol1_in1_tap20/3(coeff_out) -> pol1_in1_tap21/3(coeff)
  pol1_in1_first_tap3/1(dout) -> pol1_in1_tap19/1(din)
  pol1_in1_tap24/4(taps_out) -> delay31/1
  delay34/1 -> adder_1_4/2(din1)
  pol1_in1_tap21/5(add_out) -> pol1_in1_tap22/4(addr_in)
  delay29/1 -> adder_1_4/7(din6)
  pol1_in4_coeffs/1(dout) -> pol1_in1_first_tap3/1(din)
  delay30/1 -> adder_1_4/6(din5)
  pol1_in1_tap22/2(sync_out) -> pol1_in1_last_tap3/2(sync)
  pol1_in1_tap24/6(pot_en_out) -> pol1_in1_tap20/5(pot_en_in)
  pol1_in1_tap23/6(pot_en_out) -> pol1_in1_tap24/5(pot_en_in)
  pol1_in1_first_tap3/2(sync_out) -> pol1_in1_tap19/2(sync)
  pol1_in1_tap21/4(taps_out) -> delay29/1
  delay31/1 -> adder_1_4/5(din4)
  delay33/1 -> adder_1_4/3(din2)
  pol1_in1_tap27/3(coeff_out) -> pol1_in1_tap28/3(coeff)
  pol1_in1_tap29/5(add_out) -> pol1_in1_tap30/4(addr_in)
  pol1_in1_first_tap4/6(pot_en_out) -> pol1_in1_tap25/5(pot_en_in)
  pol1_in1_tap28/3(coeff_out) -> pol1_in1_last_tap4/3(coeff)
  pol1_in1_tap26/4(taps_out) -> delay38/1
  pol1_in1_tap27/2(sync_out) -> pol1_in1_tap28/2(sync)
  [tap_write_en] -> pol1_in1_first_tap4/5(pot_en_in)
  pol1_in1_tap30/1(dout) -> pol1_in1_tap26/1(din)
  pol1_in1_tap30/5(add_out) -> pol1_in1_tap26/4(addr_in)
  pol1_in1_tap25/6(pot_en_out) -> pol1_in1_tap29/5(pot_en_in)
  pol1_in1_tap26/5(add_out) -> pol1_in1_tap27/4(addr_in)
  pol1_in1_last_tap4/1(tap_out) -> adder_1_5/9(din8)
  pol1_in1_first_tap4/4(taps_out) -> delay42/1
  pol1_in1_tap29/1(dout) -> pol1_in1_tap30/1(din)
  pol1_in1_tap26/2(sync_out) -> pol1_in1_tap27/2(sync)
  pol1_in5_coeffs/3(coeff) -> pol1_in1_first_tap4/3(coeffs)
  pol1_in1_tap28/1(dout) -> pol1_in1_last_tap4/1(din)
  [addr] -> pol1_in1_first_tap4/4(addr_in)
  pol1_in1_tap27/1(dout) -> pol1_in1_tap28/1(din)
  pol1_in1_tap29/3(coeff_out) -> pol1_in1_tap30/3(coeff)
  pol1_in1_tap25/3(coeff_out) -> pol1_in1_tap29/3(coeff)
  pol1_in1_tap25/1(dout) -> pol1_in1_tap29/1(din)
  delay40/1 -> adder_1_5/4(din3)
  pol1_in1_tap30/3(coeff_out) -> pol1_in1_tap26/3(coeff)
  pol1_in1_tap25/5(add_out) -> pol1_in1_tap29/4(addr_in)
  pol1_in1_tap26/1(dout) -> pol1_in1_tap27/1(din)
  pol1_in1_tap26/6(pot_en_out) -> pol1_in1_tap27/5(pot_en_in)
  pol1_in1_tap29/2(sync_out) -> pol1_in1_tap30/2(sync)
  pol1_in1_tap25/2(sync_out) -> pol1_in1_tap29/2(sync)
  pol1_in1_first_tap4/3(coeff_out) -> pol1_in1_tap25/3(coeff)
  pol1_in1_last_tap4/2(sync_out) -> delay35/1
  pol1_in1_tap29/4(taps_out) -> delay40/1
  pol1_in1_tap25/4(taps_out) -> delay41/1
  pol1_in1_tap28/4(taps_out) -> delay36/1
  pol1_in1_tap27/6(pot_en_out) -> pol1_in1_tap28/5(pot_en_in)
  delay36/1 -> adder_1_5/8(din7)
  pol1_in1_first_tap4/5(add_out) -> pol1_in1_tap25/4(addr_in)
  pol1_in1_tap30/2(sync_out) -> pol1_in1_tap26/2(sync)
  delay35/1 -> adder_1_5/1(sync)
  pol1_in1_tap26/3(coeff_out) -> pol1_in1_tap27/3(coeff)
  pol1_in1_first_tap4/1(dout) -> pol1_in1_tap25/1(din)
  pol1_in1_tap30/4(taps_out) -> delay39/1
  delay42/1 -> adder_1_5/2(din1)
  pol1_in1_tap27/5(add_out) -> pol1_in1_tap28/4(addr_in)
  delay37/1 -> adder_1_5/7(din6)
  pol1_in5_coeffs/1(dout) -> pol1_in1_first_tap4/1(din)
  delay38/1 -> adder_1_5/6(din5)
  pol1_in1_tap28/2(sync_out) -> pol1_in1_last_tap4/2(sync)
  pol1_in1_tap30/6(pot_en_out) -> pol1_in1_tap26/5(pot_en_in)
  pol1_in1_tap29/6(pot_en_out) -> pol1_in1_tap30/5(pot_en_in)
  pol1_in1_first_tap4/2(sync_out) -> pol1_in1_tap25/2(sync)
  pol1_in1_tap27/4(taps_out) -> delay37/1
  delay39/1 -> adder_1_5/5(din4)
  delay41/1 -> adder_1_5/3(din2)
  pol1_in1_tap33/3(coeff_out) -> pol1_in1_tap34/3(coeff)
  pol1_in1_tap35/5(add_out) -> pol1_in1_tap36/4(addr_in)
  pol1_in1_first_tap5/6(pot_en_out) -> pol1_in1_tap31/5(pot_en_in)
  pol1_in1_tap34/3(coeff_out) -> pol1_in1_last_tap5/3(coeff)
  pol1_in1_tap32/4(taps_out) -> delay46/1
  pol1_in1_tap33/2(sync_out) -> pol1_in1_tap34/2(sync)
  [tap_write_en] -> pol1_in1_first_tap5/5(pot_en_in)
  pol1_in1_tap36/1(dout) -> pol1_in1_tap32/1(din)
  pol1_in1_tap36/5(add_out) -> pol1_in1_tap32/4(addr_in)
  pol1_in1_tap31/6(pot_en_out) -> pol1_in1_tap35/5(pot_en_in)
  pol1_in1_tap32/5(add_out) -> pol1_in1_tap33/4(addr_in)
  pol1_in1_last_tap5/1(tap_out) -> adder_1_6/9(din8)
  pol1_in1_first_tap5/4(taps_out) -> delay50/1
  pol1_in1_tap35/1(dout) -> pol1_in1_tap36/1(din)
  pol1_in1_tap32/2(sync_out) -> pol1_in1_tap33/2(sync)
  pol1_in6_coeffs/3(coeff) -> pol1_in1_first_tap5/3(coeffs)
  pol1_in1_tap34/1(dout) -> pol1_in1_last_tap5/1(din)
  [addr] -> pol1_in1_first_tap5/4(addr_in)
  pol1_in1_tap33/1(dout) -> pol1_in1_tap34/1(din)
  pol1_in1_tap35/3(coeff_out) -> pol1_in1_tap36/3(coeff)
  pol1_in1_tap31/3(coeff_out) -> pol1_in1_tap35/3(coeff)
  pol1_in1_tap31/1(dout) -> pol1_in1_tap35/1(din)
  delay48/1 -> adder_1_6/4(din3)
  pol1_in1_tap36/3(coeff_out) -> pol1_in1_tap32/3(coeff)
  pol1_in1_tap31/5(add_out) -> pol1_in1_tap35/4(addr_in)
  pol1_in1_tap32/1(dout) -> pol1_in1_tap33/1(din)
  pol1_in1_tap32/6(pot_en_out) -> pol1_in1_tap33/5(pot_en_in)
  pol1_in1_tap35/2(sync_out) -> pol1_in1_tap36/2(sync)
  pol1_in1_tap31/2(sync_out) -> pol1_in1_tap35/2(sync)
  pol1_in1_first_tap5/3(coeff_out) -> pol1_in1_tap31/3(coeff)
  pol1_in1_last_tap5/2(sync_out) -> delay43/1
  pol1_in1_tap35/4(taps_out) -> delay48/1
  pol1_in1_tap31/4(taps_out) -> delay49/1
  pol1_in1_tap34/4(taps_out) -> delay44/1
  pol1_in1_tap33/6(pot_en_out) -> pol1_in1_tap34/5(pot_en_in)
  delay44/1 -> adder_1_6/8(din7)
  pol1_in1_first_tap5/5(add_out) -> pol1_in1_tap31/4(addr_in)
  pol1_in1_tap36/2(sync_out) -> pol1_in1_tap32/2(sync)
  delay43/1 -> adder_1_6/1(sync)
  pol1_in1_tap32/3(coeff_out) -> pol1_in1_tap33/3(coeff)
  pol1_in1_first_tap5/1(dout) -> pol1_in1_tap31/1(din)
  pol1_in1_tap36/4(taps_out) -> delay47/1
  delay50/1 -> adder_1_6/2(din1)
  pol1_in1_tap33/5(add_out) -> pol1_in1_tap34/4(addr_in)
  delay45/1 -> adder_1_6/7(din6)
  pol1_in6_coeffs/1(dout) -> pol1_in1_first_tap5/1(din)
  delay46/1 -> adder_1_6/6(din5)
  pol1_in1_tap34/2(sync_out) -> pol1_in1_last_tap5/2(sync)
  pol1_in1_tap36/6(pot_en_out) -> pol1_in1_tap32/5(pot_en_in)
  pol1_in1_tap35/6(pot_en_out) -> pol1_in1_tap36/5(pot_en_in)
  pol1_in1_first_tap5/2(sync_out) -> pol1_in1_tap31/2(sync)
  pol1_in1_tap33/4(taps_out) -> delay45/1
  delay47/1 -> adder_1_6/5(din4)
  delay49/1 -> adder_1_6/3(din2)
  pol1_in1_tap39/3(coeff_out) -> pol1_in1_tap40/3(coeff)
  pol1_in1_tap41/5(add_out) -> pol1_in1_tap42/4(addr_in)
  pol1_in1_first_tap6/6(pot_en_out) -> pol1_in1_tap37/5(pot_en_in)
  pol1_in1_tap40/3(coeff_out) -> pol1_in1_last_tap6/3(coeff)
  pol1_in1_tap38/4(taps_out) -> delay54/1
  pol1_in1_tap39/2(sync_out) -> pol1_in1_tap40/2(sync)
  [tap_write_en] -> pol1_in1_first_tap6/5(pot_en_in)
  pol1_in1_tap42/1(dout) -> pol1_in1_tap38/1(din)
  pol1_in1_tap42/5(add_out) -> pol1_in1_tap38/4(addr_in)
  pol1_in1_tap37/6(pot_en_out) -> pol1_in1_tap41/5(pot_en_in)
  pol1_in1_tap38/5(add_out) -> pol1_in1_tap39/4(addr_in)
  pol1_in1_last_tap6/1(tap_out) -> adder_1_7/9(din8)
  pol1_in1_first_tap6/4(taps_out) -> delay58/1
  pol1_in1_tap41/1(dout) -> pol1_in1_tap42/1(din)
  pol1_in1_tap38/2(sync_out) -> pol1_in1_tap39/2(sync)
  pol1_in7_coeffs/3(coeff) -> pol1_in1_first_tap6/3(coeffs)
  pol1_in1_tap40/1(dout) -> pol1_in1_last_tap6/1(din)
  [addr] -> pol1_in1_first_tap6/4(addr_in)
  pol1_in1_tap39/1(dout) -> pol1_in1_tap40/1(din)
  pol1_in1_tap41/3(coeff_out) -> pol1_in1_tap42/3(coeff)
  pol1_in1_tap37/3(coeff_out) -> pol1_in1_tap41/3(coeff)
  pol1_in1_tap37/1(dout) -> pol1_in1_tap41/1(din)
  delay56/1 -> adder_1_7/4(din3)
  pol1_in1_tap42/3(coeff_out) -> pol1_in1_tap38/3(coeff)
  pol1_in1_tap37/5(add_out) -> pol1_in1_tap41/4(addr_in)
  pol1_in1_tap38/1(dout) -> pol1_in1_tap39/1(din)
  pol1_in1_tap38/6(pot_en_out) -> pol1_in1_tap39/5(pot_en_in)
  pol1_in1_tap41/2(sync_out) -> pol1_in1_tap42/2(sync)
  pol1_in1_tap37/2(sync_out) -> pol1_in1_tap41/2(sync)
  pol1_in1_first_tap6/3(coeff_out) -> pol1_in1_tap37/3(coeff)
  pol1_in1_last_tap6/2(sync_out) -> delay51/1
  pol1_in1_tap41/4(taps_out) -> delay56/1
  pol1_in1_tap37/4(taps_out) -> delay57/1
  pol1_in1_tap40/4(taps_out) -> delay52/1
  pol1_in1_tap39/6(pot_en_out) -> pol1_in1_tap40/5(pot_en_in)
  delay52/1 -> adder_1_7/8(din7)
  pol1_in1_first_tap6/5(add_out) -> pol1_in1_tap37/4(addr_in)
  pol1_in1_tap42/2(sync_out) -> pol1_in1_tap38/2(sync)
  delay51/1 -> adder_1_7/1(sync)
  pol1_in1_tap38/3(coeff_out) -> pol1_in1_tap39/3(coeff)
  pol1_in1_first_tap6/1(dout) -> pol1_in1_tap37/1(din)
  pol1_in1_tap42/4(taps_out) -> delay55/1
  delay58/1 -> adder_1_7/2(din1)
  pol1_in1_tap39/5(add_out) -> pol1_in1_tap40/4(addr_in)
  delay53/1 -> adder_1_7/7(din6)
  pol1_in7_coeffs/1(dout) -> pol1_in1_first_tap6/1(din)
  delay54/1 -> adder_1_7/6(din5)
  pol1_in1_tap40/2(sync_out) -> pol1_in1_last_tap6/2(sync)
  pol1_in1_tap42/6(pot_en_out) -> pol1_in1_tap38/5(pot_en_in)
  pol1_in1_tap41/6(pot_en_out) -> pol1_in1_tap42/5(pot_en_in)
  pol1_in1_first_tap6/2(sync_out) -> pol1_in1_tap37/2(sync)
  pol1_in1_tap39/4(taps_out) -> delay53/1
  delay55/1 -> adder_1_7/5(din4)
  delay57/1 -> adder_1_7/3(din2)
  pol1_in1_tap45/3(coeff_out) -> pol1_in1_tap46/3(coeff)
  pol1_in1_tap47/5(add_out) -> pol1_in1_tap48/4(addr_in)
  pol1_in1_first_tap7/6(pot_en_out) -> pol1_in1_tap43/5(pot_en_in)
  pol1_in1_tap46/3(coeff_out) -> pol1_in1_last_tap7/3(coeff)
  pol1_in1_tap44/4(taps_out) -> delay62/1
  pol1_in1_tap45/2(sync_out) -> pol1_in1_tap46/2(sync)
  [tap_write_en] -> pol1_in1_first_tap7/5(pot_en_in)
  pol1_in1_tap48/1(dout) -> pol1_in1_tap44/1(din)
  pol1_in1_tap48/5(add_out) -> pol1_in1_tap44/4(addr_in)
  pol1_in1_tap43/6(pot_en_out) -> pol1_in1_tap47/5(pot_en_in)
  pol1_in1_tap44/5(add_out) -> pol1_in1_tap45/4(addr_in)
  pol1_in1_last_tap7/1(tap_out) -> adder_1_8/9(din8)
  pol1_in1_first_tap7/4(taps_out) -> delay66/1
  pol1_in1_tap47/1(dout) -> pol1_in1_tap48/1(din)
  pol1_in1_tap44/2(sync_out) -> pol1_in1_tap45/2(sync)
  pol1_in8_coeffs/3(coeff) -> pol1_in1_first_tap7/3(coeffs)
  pol1_in1_tap46/1(dout) -> pol1_in1_last_tap7/1(din)
  [addr] -> pol1_in1_first_tap7/4(addr_in)
  pol1_in1_tap45/1(dout) -> pol1_in1_tap46/1(din)
  pol1_in1_tap47/3(coeff_out) -> pol1_in1_tap48/3(coeff)
  pol1_in1_tap43/3(coeff_out) -> pol1_in1_tap47/3(coeff)
  pol1_in1_tap43/1(dout) -> pol1_in1_tap47/1(din)
  delay64/1 -> adder_1_8/4(din3)
  pol1_in1_tap48/3(coeff_out) -> pol1_in1_tap44/3(coeff)
  pol1_in1_tap43/5(add_out) -> pol1_in1_tap47/4(addr_in)
  pol1_in1_tap44/1(dout) -> pol1_in1_tap45/1(din)
  pol1_in1_tap44/6(pot_en_out) -> pol1_in1_tap45/5(pot_en_in)
  pol1_in1_tap47/2(sync_out) -> pol1_in1_tap48/2(sync)
  pol1_in1_tap43/2(sync_out) -> pol1_in1_tap47/2(sync)
  pol1_in1_first_tap7/3(coeff_out) -> pol1_in1_tap43/3(coeff)
  pol1_in1_last_tap7/2(sync_out) -> delay59/1
  pol1_in1_tap47/4(taps_out) -> delay64/1
  pol1_in1_tap43/4(taps_out) -> delay65/1
  pol1_in1_tap46/4(taps_out) -> delay60/1
  pol1_in1_tap45/6(pot_en_out) -> pol1_in1_tap46/5(pot_en_in)
  delay60/1 -> adder_1_8/8(din7)
  pol1_in1_first_tap7/5(add_out) -> pol1_in1_tap43/4(addr_in)
  pol1_in1_tap48/2(sync_out) -> pol1_in1_tap44/2(sync)
  delay59/1 -> adder_1_8/1(sync)
  pol1_in1_tap44/3(coeff_out) -> pol1_in1_tap45/3(coeff)
  pol1_in1_first_tap7/1(dout) -> pol1_in1_tap43/1(din)
  pol1_in1_tap48/4(taps_out) -> delay63/1
  delay66/1 -> adder_1_8/2(din1)
  pol1_in1_tap45/5(add_out) -> pol1_in1_tap46/4(addr_in)
  delay61/1 -> adder_1_8/7(din6)
  pol1_in8_coeffs/1(dout) -> pol1_in1_first_tap7/1(din)
  delay62/1 -> adder_1_8/6(din5)
  pol1_in1_tap46/2(sync_out) -> pol1_in1_last_tap7/2(sync)
  pol1_in1_tap48/6(pot_en_out) -> pol1_in1_tap44/5(pot_en_in)
  pol1_in1_tap47/6(pot_en_out) -> pol1_in1_tap48/5(pot_en_in)
  pol1_in1_first_tap7/2(sync_out) -> pol1_in1_tap43/2(sync)
  pol1_in1_tap45/4(taps_out) -> delay61/1
  delay63/1 -> adder_1_8/5(din4)
  delay65/1 -> adder_1_8/3(din2)
  pol1_in1_tap51/3(coeff_out) -> pol1_in1_tap52/3(coeff)
  pol1_in1_tap53/5(add_out) -> pol1_in1_tap54/4(addr_in)
  pol1_in1_first_tap8/6(pot_en_out) -> pol1_in1_tap49/5(pot_en_in)
  pol1_in1_tap52/3(coeff_out) -> pol1_in1_last_tap8/3(coeff)
  pol1_in1_tap50/4(taps_out) -> delay70/1
  pol1_in1_tap51/2(sync_out) -> pol1_in1_tap52/2(sync)
  [tap_write_en] -> pol1_in1_first_tap8/5(pot_en_in)
  pol1_in1_tap54/1(dout) -> pol1_in1_tap50/1(din)
  pol1_in1_tap54/5(add_out) -> pol1_in1_tap50/4(addr_in)
  pol1_in1_tap49/6(pot_en_out) -> pol1_in1_tap53/5(pot_en_in)
  pol1_in1_tap50/5(add_out) -> pol1_in1_tap51/4(addr_in)
  pol1_in1_last_tap8/1(tap_out) -> adder_1_9/9(din8)
  pol1_in1_first_tap8/4(taps_out) -> delay74/1
  pol1_in1_tap53/1(dout) -> pol1_in1_tap54/1(din)
  pol1_in1_tap50/2(sync_out) -> pol1_in1_tap51/2(sync)
  pol1_in9_coeffs/3(coeff) -> pol1_in1_first_tap8/3(coeffs)
  pol1_in1_tap52/1(dout) -> pol1_in1_last_tap8/1(din)
  [addr] -> pol1_in1_first_tap8/4(addr_in)
  pol1_in1_tap51/1(dout) -> pol1_in1_tap52/1(din)
  pol1_in1_tap53/3(coeff_out) -> pol1_in1_tap54/3(coeff)
  pol1_in1_tap49/3(coeff_out) -> pol1_in1_tap53/3(coeff)
  pol1_in1_tap49/1(dout) -> pol1_in1_tap53/1(din)
  delay72/1 -> adder_1_9/4(din3)
  pol1_in1_tap54/3(coeff_out) -> pol1_in1_tap50/3(coeff)
  pol1_in1_tap49/5(add_out) -> pol1_in1_tap53/4(addr_in)
  pol1_in1_tap50/1(dout) -> pol1_in1_tap51/1(din)
  pol1_in1_tap50/6(pot_en_out) -> pol1_in1_tap51/5(pot_en_in)
  pol1_in1_tap53/2(sync_out) -> pol1_in1_tap54/2(sync)
  pol1_in1_tap49/2(sync_out) -> pol1_in1_tap53/2(sync)
  pol1_in1_first_tap8/3(coeff_out) -> pol1_in1_tap49/3(coeff)
  pol1_in1_last_tap8/2(sync_out) -> delay67/1
  pol1_in1_tap53/4(taps_out) -> delay72/1
  pol1_in1_tap49/4(taps_out) -> delay73/1
  pol1_in1_tap52/4(taps_out) -> delay68/1
  pol1_in1_tap51/6(pot_en_out) -> pol1_in1_tap52/5(pot_en_in)
  delay68/1 -> adder_1_9/8(din7)
  pol1_in1_first_tap8/5(add_out) -> pol1_in1_tap49/4(addr_in)
  pol1_in1_tap54/2(sync_out) -> pol1_in1_tap50/2(sync)
  delay67/1 -> adder_1_9/1(sync)
  pol1_in1_tap50/3(coeff_out) -> pol1_in1_tap51/3(coeff)
  pol1_in1_first_tap8/1(dout) -> pol1_in1_tap49/1(din)
  pol1_in1_tap54/4(taps_out) -> delay71/1
  delay74/1 -> adder_1_9/2(din1)
  pol1_in1_tap51/5(add_out) -> pol1_in1_tap52/4(addr_in)
  delay69/1 -> adder_1_9/7(din6)
  pol1_in9_coeffs/1(dout) -> pol1_in1_first_tap8/1(din)
  delay70/1 -> adder_1_9/6(din5)
  pol1_in1_tap52/2(sync_out) -> pol1_in1_last_tap8/2(sync)
  pol1_in1_tap54/6(pot_en_out) -> pol1_in1_tap50/5(pot_en_in)
  pol1_in1_tap53/6(pot_en_out) -> pol1_in1_tap54/5(pot_en_in)
  pol1_in1_first_tap8/2(sync_out) -> pol1_in1_tap49/2(sync)
  pol1_in1_tap51/4(taps_out) -> delay69/1
  delay71/1 -> adder_1_9/5(din4)
  delay73/1 -> adder_1_9/3(din2)
  pol1_in1_tap57/3(coeff_out) -> pol1_in1_tap58/3(coeff)
  pol1_in1_tap59/5(add_out) -> pol1_in1_tap60/4(addr_in)
  pol1_in1_first_tap9/6(pot_en_out) -> pol1_in1_tap55/5(pot_en_in)
  pol1_in1_tap58/3(coeff_out) -> pol1_in1_last_tap9/3(coeff)
  pol1_in1_tap56/4(taps_out) -> delay78/1
  pol1_in1_tap57/2(sync_out) -> pol1_in1_tap58/2(sync)
  [tap_write_en] -> pol1_in1_first_tap9/5(pot_en_in)
  pol1_in1_tap60/1(dout) -> pol1_in1_tap56/1(din)
  pol1_in1_tap60/5(add_out) -> pol1_in1_tap56/4(addr_in)
  pol1_in1_tap55/6(pot_en_out) -> pol1_in1_tap59/5(pot_en_in)
  pol1_in1_tap56/5(add_out) -> pol1_in1_tap57/4(addr_in)
  pol1_in1_last_tap9/1(tap_out) -> adder_1_10/9(din8)
  pol1_in1_first_tap9/4(taps_out) -> delay82/1
  pol1_in1_tap59/1(dout) -> pol1_in1_tap60/1(din)
  pol1_in1_tap56/2(sync_out) -> pol1_in1_tap57/2(sync)
  pol1_in10_coeffs/3(coeff) -> pol1_in1_first_tap9/3(coeffs)
  pol1_in1_tap58/1(dout) -> pol1_in1_last_tap9/1(din)
  [addr] -> pol1_in1_first_tap9/4(addr_in)
  pol1_in1_tap57/1(dout) -> pol1_in1_tap58/1(din)
  pol1_in1_tap59/3(coeff_out) -> pol1_in1_tap60/3(coeff)
  pol1_in1_tap55/3(coeff_out) -> pol1_in1_tap59/3(coeff)
  pol1_in1_tap55/1(dout) -> pol1_in1_tap59/1(din)
  delay80/1 -> adder_1_10/4(din3)
  pol1_in1_tap60/3(coeff_out) -> pol1_in1_tap56/3(coeff)
  pol1_in1_tap55/5(add_out) -> pol1_in1_tap59/4(addr_in)
  pol1_in1_tap56/1(dout) -> pol1_in1_tap57/1(din)
  pol1_in1_tap56/6(pot_en_out) -> pol1_in1_tap57/5(pot_en_in)
  pol1_in1_tap59/2(sync_out) -> pol1_in1_tap60/2(sync)
  pol1_in1_tap55/2(sync_out) -> pol1_in1_tap59/2(sync)
  pol1_in1_first_tap9/3(coeff_out) -> pol1_in1_tap55/3(coeff)
  pol1_in1_last_tap9/2(sync_out) -> delay75/1
  pol1_in1_tap59/4(taps_out) -> delay80/1
  pol1_in1_tap55/4(taps_out) -> delay81/1
  pol1_in1_tap58/4(taps_out) -> delay76/1
  pol1_in1_tap57/6(pot_en_out) -> pol1_in1_tap58/5(pot_en_in)
  delay76/1 -> adder_1_10/8(din7)
  pol1_in1_first_tap9/5(add_out) -> pol1_in1_tap55/4(addr_in)
  pol1_in1_tap60/2(sync_out) -> pol1_in1_tap56/2(sync)
  delay75/1 -> adder_1_10/1(sync)
  pol1_in1_tap56/3(coeff_out) -> pol1_in1_tap57/3(coeff)
  pol1_in1_first_tap9/1(dout) -> pol1_in1_tap55/1(din)
  pol1_in1_tap60/4(taps_out) -> delay79/1
  delay82/1 -> adder_1_10/2(din1)
  pol1_in1_tap57/5(add_out) -> pol1_in1_tap58/4(addr_in)
  delay77/1 -> adder_1_10/7(din6)
  pol1_in10_coeffs/1(dout) -> pol1_in1_first_tap9/1(din)
  delay78/1 -> adder_1_10/6(din5)
  pol1_in1_tap58/2(sync_out) -> pol1_in1_last_tap9/2(sync)
  pol1_in1_tap60/6(pot_en_out) -> pol1_in1_tap56/5(pot_en_in)
  pol1_in1_tap59/6(pot_en_out) -> pol1_in1_tap60/5(pot_en_in)
  pol1_in1_first_tap9/2(sync_out) -> pol1_in1_tap55/2(sync)
  pol1_in1_tap57/4(taps_out) -> delay77/1
  delay79/1 -> adder_1_10/5(din4)
  delay81/1 -> adder_1_10/3(din2)
  pol1_in1_tap63/3(coeff_out) -> pol1_in1_tap64/3(coeff)
  pol1_in1_tap65/5(add_out) -> pol1_in1_tap66/4(addr_in)
  pol1_in1_first_tap10/6(pot_en_out) -> pol1_in1_tap61/5(pot_en_in)
  pol1_in1_tap64/3(coeff_out) -> pol1_in1_last_tap10/3(coeff)
  pol1_in1_tap62/4(taps_out) -> delay86/1
  pol1_in1_tap63/2(sync_out) -> pol1_in1_tap64/2(sync)
  [tap_write_en] -> pol1_in1_first_tap10/5(pot_en_in)
  pol1_in1_tap66/1(dout) -> pol1_in1_tap62/1(din)
  pol1_in1_tap66/5(add_out) -> pol1_in1_tap62/4(addr_in)
  pol1_in1_tap61/6(pot_en_out) -> pol1_in1_tap65/5(pot_en_in)
  pol1_in1_tap62/5(add_out) -> pol1_in1_tap63/4(addr_in)
  pol1_in1_last_tap10/1(tap_out) -> adder_1_11/9(din8)
  pol1_in1_first_tap10/4(taps_out) -> delay90/1
  pol1_in1_tap65/1(dout) -> pol1_in1_tap66/1(din)
  pol1_in1_tap62/2(sync_out) -> pol1_in1_tap63/2(sync)
  pol1_in11_coeffs/3(coeff) -> pol1_in1_first_tap10/3(coeffs)
  pol1_in1_tap64/1(dout) -> pol1_in1_last_tap10/1(din)
  [addr] -> pol1_in1_first_tap10/4(addr_in)
  pol1_in1_tap63/1(dout) -> pol1_in1_tap64/1(din)
  pol1_in1_tap65/3(coeff_out) -> pol1_in1_tap66/3(coeff)
  pol1_in1_tap61/3(coeff_out) -> pol1_in1_tap65/3(coeff)
  pol1_in1_tap61/1(dout) -> pol1_in1_tap65/1(din)
  delay88/1 -> adder_1_11/4(din3)
  pol1_in1_tap66/3(coeff_out) -> pol1_in1_tap62/3(coeff)
  pol1_in1_tap61/5(add_out) -> pol1_in1_tap65/4(addr_in)
  pol1_in1_tap62/1(dout) -> pol1_in1_tap63/1(din)
  pol1_in1_tap62/6(pot_en_out) -> pol1_in1_tap63/5(pot_en_in)
  pol1_in1_tap65/2(sync_out) -> pol1_in1_tap66/2(sync)
  pol1_in1_tap61/2(sync_out) -> pol1_in1_tap65/2(sync)
  pol1_in1_first_tap10/3(coeff_out) -> pol1_in1_tap61/3(coeff)
  pol1_in1_last_tap10/2(sync_out) -> delay83/1
  pol1_in1_tap65/4(taps_out) -> delay88/1
  pol1_in1_tap61/4(taps_out) -> delay89/1
  pol1_in1_tap64/4(taps_out) -> delay84/1
  pol1_in1_tap63/6(pot_en_out) -> pol1_in1_tap64/5(pot_en_in)
  delay84/1 -> adder_1_11/8(din7)
  pol1_in1_first_tap10/5(add_out) -> pol1_in1_tap61/4(addr_in)
  pol1_in1_tap66/2(sync_out) -> pol1_in1_tap62/2(sync)
  delay83/1 -> adder_1_11/1(sync)
  pol1_in1_tap62/3(coeff_out) -> pol1_in1_tap63/3(coeff)
  pol1_in1_first_tap10/1(dout) -> pol1_in1_tap61/1(din)
  pol1_in1_tap66/4(taps_out) -> delay87/1
  delay90/1 -> adder_1_11/2(din1)
  pol1_in1_tap63/5(add_out) -> pol1_in1_tap64/4(addr_in)
  delay85/1 -> adder_1_11/7(din6)
  pol1_in11_coeffs/1(dout) -> pol1_in1_first_tap10/1(din)
  delay86/1 -> adder_1_11/6(din5)
  pol1_in1_tap64/2(sync_out) -> pol1_in1_last_tap10/2(sync)
  pol1_in1_tap66/6(pot_en_out) -> pol1_in1_tap62/5(pot_en_in)
  pol1_in1_tap65/6(pot_en_out) -> pol1_in1_tap66/5(pot_en_in)
  pol1_in1_first_tap10/2(sync_out) -> pol1_in1_tap61/2(sync)
  pol1_in1_tap63/4(taps_out) -> delay85/1
  delay87/1 -> adder_1_11/5(din4)
  delay89/1 -> adder_1_11/3(din2)
  pol1_in1_tap69/3(coeff_out) -> pol1_in1_tap70/3(coeff)
  pol1_in1_tap71/5(add_out) -> pol1_in1_tap72/4(addr_in)
  pol1_in1_first_tap11/6(pot_en_out) -> pol1_in1_tap67/5(pot_en_in)
  pol1_in1_tap70/3(coeff_out) -> pol1_in1_last_tap11/3(coeff)
  pol1_in1_tap68/4(taps_out) -> delay94/1
  pol1_in1_tap69/2(sync_out) -> pol1_in1_tap70/2(sync)
  [tap_write_en] -> pol1_in1_first_tap11/5(pot_en_in)
  pol1_in1_tap72/1(dout) -> pol1_in1_tap68/1(din)
  pol1_in1_tap72/5(add_out) -> pol1_in1_tap68/4(addr_in)
  pol1_in1_tap67/6(pot_en_out) -> pol1_in1_tap71/5(pot_en_in)
  pol1_in1_tap68/5(add_out) -> pol1_in1_tap69/4(addr_in)
  pol1_in1_last_tap11/1(tap_out) -> adder_1_12/9(din8)
  pol1_in1_first_tap11/4(taps_out) -> delay98/1
  pol1_in1_tap71/1(dout) -> pol1_in1_tap72/1(din)
  pol1_in1_tap68/2(sync_out) -> pol1_in1_tap69/2(sync)
  pol1_in12_coeffs/3(coeff) -> pol1_in1_first_tap11/3(coeffs)
  pol1_in1_tap70/1(dout) -> pol1_in1_last_tap11/1(din)
  [addr] -> pol1_in1_first_tap11/4(addr_in)
  pol1_in1_tap69/1(dout) -> pol1_in1_tap70/1(din)
  pol1_in1_tap71/3(coeff_out) -> pol1_in1_tap72/3(coeff)
  pol1_in1_tap67/3(coeff_out) -> pol1_in1_tap71/3(coeff)
  pol1_in1_tap67/1(dout) -> pol1_in1_tap71/1(din)
  delay96/1 -> adder_1_12/4(din3)
  pol1_in1_tap72/3(coeff_out) -> pol1_in1_tap68/3(coeff)
  pol1_in1_tap67/5(add_out) -> pol1_in1_tap71/4(addr_in)
  pol1_in1_tap68/1(dout) -> pol1_in1_tap69/1(din)
  pol1_in1_tap68/6(pot_en_out) -> pol1_in1_tap69/5(pot_en_in)
  pol1_in1_tap71/2(sync_out) -> pol1_in1_tap72/2(sync)
  pol1_in1_tap67/2(sync_out) -> pol1_in1_tap71/2(sync)
  pol1_in1_first_tap11/3(coeff_out) -> pol1_in1_tap67/3(coeff)
  pol1_in1_last_tap11/2(sync_out) -> delay91/1
  pol1_in1_tap71/4(taps_out) -> delay96/1
  pol1_in1_tap67/4(taps_out) -> delay97/1
  pol1_in1_tap70/4(taps_out) -> delay92/1
  pol1_in1_tap69/6(pot_en_out) -> pol1_in1_tap70/5(pot_en_in)
  delay92/1 -> adder_1_12/8(din7)
  pol1_in1_first_tap11/5(add_out) -> pol1_in1_tap67/4(addr_in)
  pol1_in1_tap72/2(sync_out) -> pol1_in1_tap68/2(sync)
  delay91/1 -> adder_1_12/1(sync)
  pol1_in1_tap68/3(coeff_out) -> pol1_in1_tap69/3(coeff)
  pol1_in1_first_tap11/1(dout) -> pol1_in1_tap67/1(din)
  pol1_in1_tap72/4(taps_out) -> delay95/1
  delay98/1 -> adder_1_12/2(din1)
  pol1_in1_tap69/5(add_out) -> pol1_in1_tap70/4(addr_in)
  delay93/1 -> adder_1_12/7(din6)
  pol1_in12_coeffs/1(dout) -> pol1_in1_first_tap11/1(din)
  delay94/1 -> adder_1_12/6(din5)
  pol1_in1_tap70/2(sync_out) -> pol1_in1_last_tap11/2(sync)
  pol1_in1_tap72/6(pot_en_out) -> pol1_in1_tap68/5(pot_en_in)
  pol1_in1_tap71/6(pot_en_out) -> pol1_in1_tap72/5(pot_en_in)
  pol1_in1_first_tap11/2(sync_out) -> pol1_in1_tap67/2(sync)
  pol1_in1_tap69/4(taps_out) -> delay93/1
  delay95/1 -> adder_1_12/5(din4)
  delay97/1 -> adder_1_12/3(din2)
  pol1_in1_tap75/3(coeff_out) -> pol1_in1_tap76/3(coeff)
  pol1_in1_tap77/5(add_out) -> pol1_in1_tap78/4(addr_in)
  pol1_in1_first_tap12/6(pot_en_out) -> pol1_in1_tap73/5(pot_en_in)
  pol1_in1_tap76/3(coeff_out) -> pol1_in1_last_tap12/3(coeff)
  pol1_in1_tap74/4(taps_out) -> delay102/1
  pol1_in1_tap75/2(sync_out) -> pol1_in1_tap76/2(sync)
  [tap_write_en] -> pol1_in1_first_tap12/5(pot_en_in)
  pol1_in1_tap78/1(dout) -> pol1_in1_tap74/1(din)
  pol1_in1_tap78/5(add_out) -> pol1_in1_tap74/4(addr_in)
  pol1_in1_tap73/6(pot_en_out) -> pol1_in1_tap77/5(pot_en_in)
  pol1_in1_tap74/5(add_out) -> pol1_in1_tap75/4(addr_in)
  pol1_in1_last_tap12/1(tap_out) -> adder_1_13/9(din8)
  pol1_in1_first_tap12/4(taps_out) -> delay106/1
  pol1_in1_tap77/1(dout) -> pol1_in1_tap78/1(din)
  pol1_in1_tap74/2(sync_out) -> pol1_in1_tap75/2(sync)
  pol1_in13_coeffs/3(coeff) -> pol1_in1_first_tap12/3(coeffs)
  pol1_in1_tap76/1(dout) -> pol1_in1_last_tap12/1(din)
  [addr] -> pol1_in1_first_tap12/4(addr_in)
  pol1_in1_tap75/1(dout) -> pol1_in1_tap76/1(din)
  pol1_in1_tap77/3(coeff_out) -> pol1_in1_tap78/3(coeff)
  pol1_in1_tap73/3(coeff_out) -> pol1_in1_tap77/3(coeff)
  pol1_in1_tap73/1(dout) -> pol1_in1_tap77/1(din)
  delay104/1 -> adder_1_13/4(din3)
  pol1_in1_tap78/3(coeff_out) -> pol1_in1_tap74/3(coeff)
  pol1_in1_tap73/5(add_out) -> pol1_in1_tap77/4(addr_in)
  pol1_in1_tap74/1(dout) -> pol1_in1_tap75/1(din)
  pol1_in1_tap74/6(pot_en_out) -> pol1_in1_tap75/5(pot_en_in)
  pol1_in1_tap77/2(sync_out) -> pol1_in1_tap78/2(sync)
  pol1_in1_tap73/2(sync_out) -> pol1_in1_tap77/2(sync)
  pol1_in1_first_tap12/3(coeff_out) -> pol1_in1_tap73/3(coeff)
  pol1_in1_last_tap12/2(sync_out) -> delay99/1
  pol1_in1_tap77/4(taps_out) -> delay104/1
  pol1_in1_tap73/4(taps_out) -> delay105/1
  pol1_in1_tap76/4(taps_out) -> delay100/1
  pol1_in1_tap75/6(pot_en_out) -> pol1_in1_tap76/5(pot_en_in)
  delay100/1 -> adder_1_13/8(din7)
  pol1_in1_first_tap12/5(add_out) -> pol1_in1_tap73/4(addr_in)
  pol1_in1_tap78/2(sync_out) -> pol1_in1_tap74/2(sync)
  delay99/1 -> adder_1_13/1(sync)
  pol1_in1_tap74/3(coeff_out) -> pol1_in1_tap75/3(coeff)
  pol1_in1_first_tap12/1(dout) -> pol1_in1_tap73/1(din)
  pol1_in1_tap78/4(taps_out) -> delay103/1
  delay106/1 -> adder_1_13/2(din1)
  pol1_in1_tap75/5(add_out) -> pol1_in1_tap76/4(addr_in)
  delay101/1 -> adder_1_13/7(din6)
  pol1_in13_coeffs/1(dout) -> pol1_in1_first_tap12/1(din)
  delay102/1 -> adder_1_13/6(din5)
  pol1_in1_tap76/2(sync_out) -> pol1_in1_last_tap12/2(sync)
  pol1_in1_tap78/6(pot_en_out) -> pol1_in1_tap74/5(pot_en_in)
  pol1_in1_tap77/6(pot_en_out) -> pol1_in1_tap78/5(pot_en_in)
  pol1_in1_first_tap12/2(sync_out) -> pol1_in1_tap73/2(sync)
  pol1_in1_tap75/4(taps_out) -> delay101/1
  delay103/1 -> adder_1_13/5(din4)
  delay105/1 -> adder_1_13/3(din2)
  pol1_in1_tap81/3(coeff_out) -> pol1_in1_tap82/3(coeff)
  pol1_in1_tap83/5(add_out) -> pol1_in1_tap84/4(addr_in)
  pol1_in1_first_tap13/6(pot_en_out) -> pol1_in1_tap79/5(pot_en_in)
  pol1_in1_tap82/3(coeff_out) -> pol1_in1_last_tap13/3(coeff)
  pol1_in1_tap80/4(taps_out) -> delay110/1
  pol1_in1_tap81/2(sync_out) -> pol1_in1_tap82/2(sync)
  [tap_write_en] -> pol1_in1_first_tap13/5(pot_en_in)
  pol1_in1_tap84/1(dout) -> pol1_in1_tap80/1(din)
  pol1_in1_tap84/5(add_out) -> pol1_in1_tap80/4(addr_in)
  pol1_in1_tap79/6(pot_en_out) -> pol1_in1_tap83/5(pot_en_in)
  pol1_in1_tap80/5(add_out) -> pol1_in1_tap81/4(addr_in)
  pol1_in1_last_tap13/1(tap_out) -> adder_1_14/9(din8)
  pol1_in1_first_tap13/4(taps_out) -> delay114/1
  pol1_in1_tap83/1(dout) -> pol1_in1_tap84/1(din)
  pol1_in1_tap80/2(sync_out) -> pol1_in1_tap81/2(sync)
  pol1_in14_coeffs/3(coeff) -> pol1_in1_first_tap13/3(coeffs)
  pol1_in1_tap82/1(dout) -> pol1_in1_last_tap13/1(din)
  [addr] -> pol1_in1_first_tap13/4(addr_in)
  pol1_in1_tap81/1(dout) -> pol1_in1_tap82/1(din)
  pol1_in1_tap83/3(coeff_out) -> pol1_in1_tap84/3(coeff)
  pol1_in1_tap79/3(coeff_out) -> pol1_in1_tap83/3(coeff)
  pol1_in1_tap79/1(dout) -> pol1_in1_tap83/1(din)
  delay112/1 -> adder_1_14/4(din3)
  pol1_in1_tap84/3(coeff_out) -> pol1_in1_tap80/3(coeff)
  pol1_in1_tap79/5(add_out) -> pol1_in1_tap83/4(addr_in)
  pol1_in1_tap80/1(dout) -> pol1_in1_tap81/1(din)
  pol1_in1_tap80/6(pot_en_out) -> pol1_in1_tap81/5(pot_en_in)
  pol1_in1_tap83/2(sync_out) -> pol1_in1_tap84/2(sync)
  pol1_in1_tap79/2(sync_out) -> pol1_in1_tap83/2(sync)
  pol1_in1_first_tap13/3(coeff_out) -> pol1_in1_tap79/3(coeff)
  pol1_in1_last_tap13/2(sync_out) -> delay107/1
  pol1_in1_tap83/4(taps_out) -> delay112/1
  pol1_in1_tap79/4(taps_out) -> delay113/1
  pol1_in1_tap82/4(taps_out) -> delay108/1
  pol1_in1_tap81/6(pot_en_out) -> pol1_in1_tap82/5(pot_en_in)
  delay108/1 -> adder_1_14/8(din7)
  pol1_in1_first_tap13/5(add_out) -> pol1_in1_tap79/4(addr_in)
  pol1_in1_tap84/2(sync_out) -> pol1_in1_tap80/2(sync)
  delay107/1 -> adder_1_14/1(sync)
  pol1_in1_tap80/3(coeff_out) -> pol1_in1_tap81/3(coeff)
  pol1_in1_first_tap13/1(dout) -> pol1_in1_tap79/1(din)
  pol1_in1_tap84/4(taps_out) -> delay111/1
  delay114/1 -> adder_1_14/2(din1)
  pol1_in1_tap81/5(add_out) -> pol1_in1_tap82/4(addr_in)
  delay109/1 -> adder_1_14/7(din6)
  pol1_in14_coeffs/1(dout) -> pol1_in1_first_tap13/1(din)
  delay110/1 -> adder_1_14/6(din5)
  pol1_in1_tap82/2(sync_out) -> pol1_in1_last_tap13/2(sync)
  pol1_in1_tap84/6(pot_en_out) -> pol1_in1_tap80/5(pot_en_in)
  pol1_in1_tap83/6(pot_en_out) -> pol1_in1_tap84/5(pot_en_in)
  pol1_in1_first_tap13/2(sync_out) -> pol1_in1_tap79/2(sync)
  pol1_in1_tap81/4(taps_out) -> delay109/1
  delay111/1 -> adder_1_14/5(din4)
  delay113/1 -> adder_1_14/3(din2)
  pol1_in1_tap87/3(coeff_out) -> pol1_in1_tap88/3(coeff)
  pol1_in1_tap89/5(add_out) -> pol1_in1_tap90/4(addr_in)
  pol1_in1_first_tap14/6(pot_en_out) -> pol1_in1_tap85/5(pot_en_in)
  pol1_in1_tap88/3(coeff_out) -> pol1_in1_last_tap14/3(coeff)
  pol1_in1_tap86/4(taps_out) -> delay118/1
  pol1_in1_tap87/2(sync_out) -> pol1_in1_tap88/2(sync)
  [tap_write_en] -> pol1_in1_first_tap14/5(pot_en_in)
  pol1_in1_tap90/1(dout) -> pol1_in1_tap86/1(din)
  pol1_in1_tap90/5(add_out) -> pol1_in1_tap86/4(addr_in)
  pol1_in1_tap85/6(pot_en_out) -> pol1_in1_tap89/5(pot_en_in)
  pol1_in1_tap86/5(add_out) -> pol1_in1_tap87/4(addr_in)
  pol1_in1_last_tap14/1(tap_out) -> adder_1_15/9(din8)
  pol1_in1_first_tap14/4(taps_out) -> delay122/1
  pol1_in1_tap89/1(dout) -> pol1_in1_tap90/1(din)
  pol1_in1_tap86/2(sync_out) -> pol1_in1_tap87/2(sync)
  pol1_in15_coeffs/3(coeff) -> pol1_in1_first_tap14/3(coeffs)
  pol1_in1_tap88/1(dout) -> pol1_in1_last_tap14/1(din)
  [addr] -> pol1_in1_first_tap14/4(addr_in)
  pol1_in1_tap87/1(dout) -> pol1_in1_tap88/1(din)
  pol1_in1_tap89/3(coeff_out) -> pol1_in1_tap90/3(coeff)
  pol1_in1_tap85/3(coeff_out) -> pol1_in1_tap89/3(coeff)
  pol1_in1_tap85/1(dout) -> pol1_in1_tap89/1(din)
  delay120/1 -> adder_1_15/4(din3)
  pol1_in1_tap90/3(coeff_out) -> pol1_in1_tap86/3(coeff)
  pol1_in1_tap85/5(add_out) -> pol1_in1_tap89/4(addr_in)
  pol1_in1_tap86/1(dout) -> pol1_in1_tap87/1(din)
  pol1_in1_tap86/6(pot_en_out) -> pol1_in1_tap87/5(pot_en_in)
  pol1_in1_tap89/2(sync_out) -> pol1_in1_tap90/2(sync)
  pol1_in1_tap85/2(sync_out) -> pol1_in1_tap89/2(sync)
  pol1_in1_first_tap14/3(coeff_out) -> pol1_in1_tap85/3(coeff)
  pol1_in1_last_tap14/2(sync_out) -> delay115/1
  pol1_in1_tap89/4(taps_out) -> delay120/1
  pol1_in1_tap85/4(taps_out) -> delay121/1
  pol1_in1_tap88/4(taps_out) -> delay116/1
  pol1_in1_tap87/6(pot_en_out) -> pol1_in1_tap88/5(pot_en_in)
  delay116/1 -> adder_1_15/8(din7)
  pol1_in1_first_tap14/5(add_out) -> pol1_in1_tap85/4(addr_in)
  pol1_in1_tap90/2(sync_out) -> pol1_in1_tap86/2(sync)
  delay115/1 -> adder_1_15/1(sync)
  pol1_in1_tap86/3(coeff_out) -> pol1_in1_tap87/3(coeff)
  pol1_in1_first_tap14/1(dout) -> pol1_in1_tap85/1(din)
  pol1_in1_tap90/4(taps_out) -> delay119/1
  delay122/1 -> adder_1_15/2(din1)
  pol1_in1_tap87/5(add_out) -> pol1_in1_tap88/4(addr_in)
  delay117/1 -> adder_1_15/7(din6)
  pol1_in15_coeffs/1(dout) -> pol1_in1_first_tap14/1(din)
  delay118/1 -> adder_1_15/6(din5)
  pol1_in1_tap88/2(sync_out) -> pol1_in1_last_tap14/2(sync)
  pol1_in1_tap90/6(pot_en_out) -> pol1_in1_tap86/5(pot_en_in)
  pol1_in1_tap89/6(pot_en_out) -> pol1_in1_tap90/5(pot_en_in)
  pol1_in1_first_tap14/2(sync_out) -> pol1_in1_tap85/2(sync)
  pol1_in1_tap87/4(taps_out) -> delay117/1
  delay119/1 -> adder_1_15/5(din4)
  delay121/1 -> adder_1_15/3(din2)
  pol1_in1_tap93/3(coeff_out) -> pol1_in1_tap94/3(coeff)
  pol1_in1_tap95/5(add_out) -> pol1_in1_tap96/4(addr_in)
  pol1_in1_first_tap15/6(pot_en_out) -> pol1_in1_tap91/5(pot_en_in)
  pol1_in1_tap94/3(coeff_out) -> pol1_in1_last_tap15/3(coeff)
  pol1_in1_tap92/4(taps_out) -> delay126/1
  pol1_in1_tap93/2(sync_out) -> pol1_in1_tap94/2(sync)
  [tap_write_en] -> pol1_in1_first_tap15/5(pot_en_in)
  pol1_in1_tap96/1(dout) -> pol1_in1_tap92/1(din)
  pol1_in1_tap96/5(add_out) -> pol1_in1_tap92/4(addr_in)
  pol1_in1_tap91/6(pot_en_out) -> pol1_in1_tap95/5(pot_en_in)
  pol1_in1_tap92/5(add_out) -> pol1_in1_tap93/4(addr_in)
  pol1_in1_last_tap15/1(tap_out) -> adder_1_16/9(din8)
  pol1_in1_first_tap15/4(taps_out) -> delay130/1
  pol1_in1_tap95/1(dout) -> pol1_in1_tap96/1(din)
  pol1_in1_tap92/2(sync_out) -> pol1_in1_tap93/2(sync)
  pol1_in16_coeffs/3(coeff) -> pol1_in1_first_tap15/3(coeffs)
  pol1_in1_tap94/1(dout) -> pol1_in1_last_tap15/1(din)
  [addr] -> pol1_in1_first_tap15/4(addr_in)
  pol1_in1_tap93/1(dout) -> pol1_in1_tap94/1(din)
  pol1_in1_tap95/3(coeff_out) -> pol1_in1_tap96/3(coeff)
  pol1_in1_tap91/3(coeff_out) -> pol1_in1_tap95/3(coeff)
  pol1_in1_tap91/1(dout) -> pol1_in1_tap95/1(din)
  delay128/1 -> adder_1_16/4(din3)
  pol1_in1_tap96/3(coeff_out) -> pol1_in1_tap92/3(coeff)
  pol1_in1_tap91/5(add_out) -> pol1_in1_tap95/4(addr_in)
  pol1_in1_tap92/1(dout) -> pol1_in1_tap93/1(din)
  pol1_in1_tap92/6(pot_en_out) -> pol1_in1_tap93/5(pot_en_in)
  pol1_in1_tap95/2(sync_out) -> pol1_in1_tap96/2(sync)
  pol1_in1_tap91/2(sync_out) -> pol1_in1_tap95/2(sync)
  pol1_in1_first_tap15/3(coeff_out) -> pol1_in1_tap91/3(coeff)
  pol1_in1_last_tap15/2(sync_out) -> delay123/1
  pol1_in1_tap95/4(taps_out) -> delay128/1
  pol1_in1_tap91/4(taps_out) -> delay129/1
  pol1_in1_tap94/4(taps_out) -> delay124/1
  pol1_in1_tap93/6(pot_en_out) -> pol1_in1_tap94/5(pot_en_in)
  delay124/1 -> adder_1_16/8(din7)
  pol1_in1_first_tap15/5(add_out) -> pol1_in1_tap91/4(addr_in)
  pol1_in1_tap96/2(sync_out) -> pol1_in1_tap92/2(sync)
  delay123/1 -> adder_1_16/1(sync)
  pol1_in1_tap92/3(coeff_out) -> pol1_in1_tap93/3(coeff)
  pol1_in1_first_tap15/1(dout) -> pol1_in1_tap91/1(din)
  pol1_in1_tap96/4(taps_out) -> delay127/1
  delay130/1 -> adder_1_16/2(din1)
  pol1_in1_tap93/5(add_out) -> pol1_in1_tap94/4(addr_in)
  delay125/1 -> adder_1_16/7(din6)
  pol1_in16_coeffs/1(dout) -> pol1_in1_first_tap15/1(din)
  delay126/1 -> adder_1_16/6(din5)
  pol1_in1_tap94/2(sync_out) -> pol1_in1_last_tap15/2(sync)
  pol1_in1_tap96/6(pot_en_out) -> pol1_in1_tap92/5(pot_en_in)
  pol1_in1_tap95/6(pot_en_out) -> pol1_in1_tap96/5(pot_en_in)
  pol1_in1_first_tap15/2(sync_out) -> pol1_in1_tap91/2(sync)
  pol1_in1_tap93/4(taps_out) -> delay125/1
  delay127/1 -> adder_1_16/5(din4)
  delay129/1 -> adder_1_16/3(din2)
  pol1_in2_coeffs/2(sync_out) -> pol1_in1_first_tap1/2(sync)
  pol1_in3_coeffs/2(sync_out) -> pol1_in1_first_tap2/2(sync)
  pol1_in4_coeffs/2(sync_out) -> pol1_in1_first_tap3/2(sync)
  pol1_in5_coeffs/2(sync_out) -> pol1_in1_first_tap4/2(sync)
  pol1_in6_coeffs/2(sync_out) -> pol1_in1_first_tap5/2(sync)
  pol1_in7_coeffs/2(sync_out) -> pol1_in1_first_tap6/2(sync)
  pol1_in8_coeffs/2(sync_out) -> pol1_in1_first_tap7/2(sync)
  pol1_in9_coeffs/2(sync_out) -> pol1_in1_first_tap8/2(sync)
  pol1_in10_coeffs/2(sync_out) -> pol1_in1_first_tap9/2(sync)
  pol1_in11_coeffs/2(sync_out) -> pol1_in1_first_tap10/2(sync)
  pol1_in12_coeffs/2(sync_out) -> pol1_in1_first_tap11/2(sync)
  pol1_in13_coeffs/2(sync_out) -> pol1_in1_first_tap12/2(sync)
  pol1_in14_coeffs/2(sync_out) -> pol1_in1_first_tap13/2(sync)
  pol1_in15_coeffs/2(sync_out) -> pol1_in1_first_tap14/2(sync)
  pol1_in16_coeffs/2(sync_out) -> pol1_in1_first_tap15/2(sync)
